simulink model "FullFMS_2026_02_18_V0_3_9"  (R2025b)
settings: Solver=ode23tb  StartTime=0.0  StopTime=inf  MaxStep=0.1  RelTol=1e-2
PreLoadFcn:
  | load("BUS_CONFIG.mat")
libraries: opcualib x8
(part 1 of 4)
settings Model: SimulationMode=accelerator  PacingRate=0.100000  Creator=guilh  LastModifiedBy=guilh
settings SolverCC: ZeroCrossControl=DisableAll

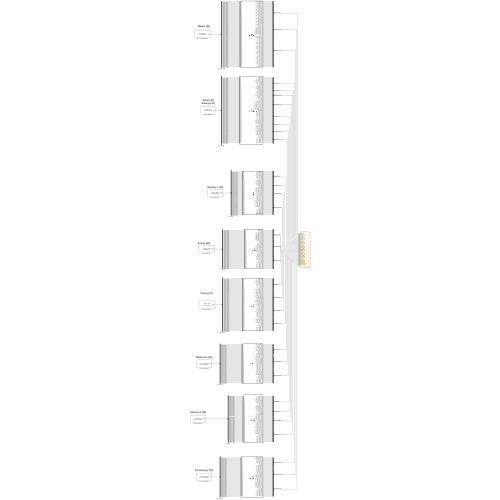
[thumbnail: Simulink's stored preview of the top-level diagram]
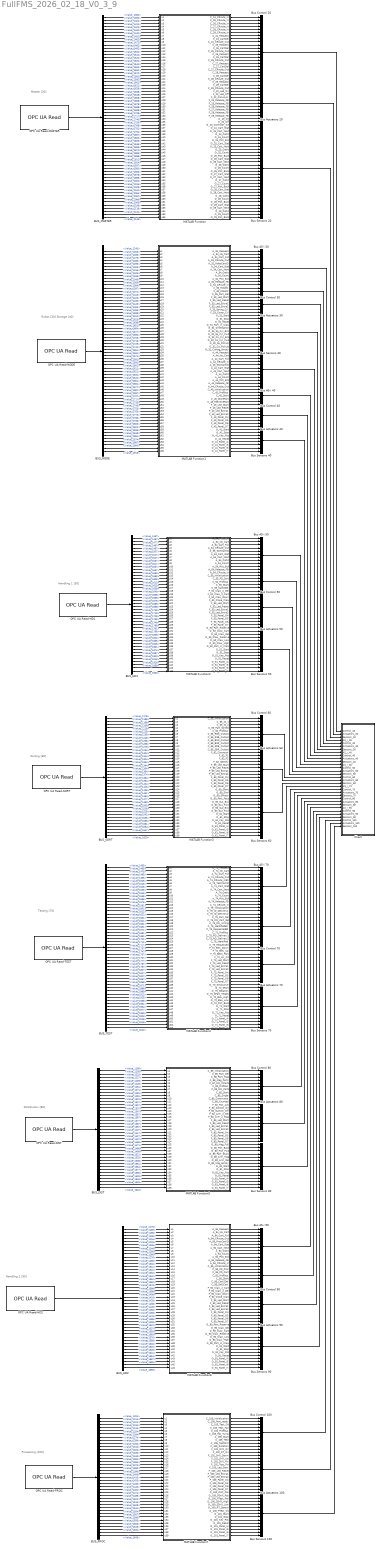
== system FullFMS_2026_02_18_V0_3_9 ==
  note: Master [20]
  note: Robot [30]
      | Storage [40]
  note: Handling 1 [50]
  note: Sorting [60]
  note: Testing [70]
  note: Distribution [80]
  note: Handling 2 [90]
  note: Processing [100]
  BUS_DIST : BusSelector  OutputSignals=Value_1195,Value_1205,Value_1215,Value_1227,Value_1239,Value_1249,Value_1261,Value_1271,Value_1281,Value_1291,Value_1301,Value_1317,Value_1327,Value_1337,Value_1347,Value_1357,Value_1367,Value_1377,Value_1387,Value_1397,Value_1407,Value_1417,Value_1427,Value_1437,Value_1458,Value_1471,Value_1486,Value_1499,Value_1512,Value_1525,Value_1538,Value_1551,Value_1564,Value_1577,Value_1590,Value_1603,Value_1616,Value_1629,Value_1642
  BUS_HD1 : BusSelector  OutputSignals=Value_1457,Value_1467,Value_1477,Value_1487,Value_1497,Value_1507,Value_1517,Value_1527,Value_1537,Value_1547,Value_1557,Value_1567,Value_1583,Value_1593,Value_1603,Value_1613,Value_1623,Value_1639,Value_1649,Value_1659,Value_1669,Value_1679,Value_1689,Value_1699,Value_1709,Value_1719,Value_1729,Value_1739,Value_1749,Value_1768,Value_1781,Value_1796,Value_1809,Value_1822,Value_1835,Value_1848,Value_1861,Value_1874,Value_1887,Value_1900,Value_1913,Value_1926,Value_1939,Value_1952
  BUS_HD2 : BusSelector  OutputSignals=Value_1176,Value_1186,Value_1196,Value_1206,Value_1216,Value_1226,Value_1236,Value_1246,Value_1256,Value_1266,Value_1276,Value_1286,Value_1302,Value_1312,Value_1322,Value_1332,Value_1342,Value_1352,Value_1362,Value_1378,Value_1388,Value_1398,Value_1408,Value_1418,Value_1428,Value_1438,Value_1448,Value_1458,Value_1468,Value_1478,Value_1488,Value_1509,Value_1522,Value_1537,Value_1550,Value_1563,Value_1576,Value_1589,Value_1602,Value_1615,Value_1628,Value_1641,Value_1654,Value_1667,Value_1680,Value_1693
  BUS_MASTER : BusSelector  OutputSignals=Value_1382,Value_1392,Value_1402,Value_1412,Value_1422,Value_1432,Value_1442,Value_1452,Value_1462,Value_1472,Value_1482,Value_1492,Value_1502,Value_1512,Value_1522,Value_1532,Value_1542,Value_1552,Value_1562,Value_1572,Value_1582,Value_1592,Value_1602,Value_1612,Value_1628,Value_1638,Value_1648,Value_1658,Value_1668,Value_1678,Value_1688,Value_1698,Value_1708,Value_1727,Value_1740,Value_1755,Value_1768,Value_1781,Value_1794,Value_1807,Value_1820,Value_1833,Value_1846,Value_1859,Value_1872,Value_1885,Value_1898,Value_1911,Value_1924,Value_1937,Value_1950,Value_1963,Value_1976,Value_1989,Value_2002,Value_2015,Value_2028,Value_2041,Value_2054,Value_2067,Value_2080,Value_2093,Value_2106,Value_2119,Value_2132,Value_2145
  BUS_NODE : BusSelector  OutputSignals=Value_1245,Value_1255,Value_1265,Value_1275,Value_1285,Value_1295,Value_1305,Value_1315,Value_1325,Value_1335,Value_1345,Value_1355,Value_1384,Value_1397,Value_1371,Value_1413,Value_1423,Value_1433,Value_1443,Value_1453,Value_1463,Value_1599,Value_1612,Value_1625,Value_1638,Value_1651,Value_1664,Value_1677,Value_1690,Value_1703,Value_1716,Value_1729,Value_1742,Value_2551,Value_2561,Value_2571,Value_2581,Value_2591,Value_2601,Value_2611,Value_2621,Value_2631,Value_2641,Value_2651,Value_2661,Value_2677,Value_2687,Value_2697,Value_2707,Value_2717,Value_2733,Value_2743,Value_2753,Value_2763,Value_2773,Value_2783,Value_2793,Value_2803,Value_2822,Value_2835,Value_2848,Value_2861,Value_2874,Value_2887,Value_2900,Value_2913
  BUS_PROC : BusSelector  OutputSignals=Value_1204,Value_1214,Value_1224,Value_1234,Value_1244,Value_1254,Value_1264,Value_1274,Value_1284,Value_1294,Value_1310,Value_1320,Value_1330,Value_1340,Value_1350,Value_1360,Value_1370,Value_1380,Value_1390,Value_1400,Value_1410,Value_1420,Value_1430,Value_1440,Value_1461,Value_1474,Value_1489,Value_1502,Value_1515,Value_1528,Value_1541,Value_1554,Value_1567,Value_1580,Value_1593,Value_1606,Value_1619,Value_1632,Value_1645
  BUS_SORT : BusSelector  OutputSignals=Value_1178,Value_1188,Value_1198,Value_1208,Value_1218,Value_1228,Value_1238,Value_1248,Value_1258,Value_1268,Value_1278,Value_1294,Value_1304,Value_1314,Value_1324,Value_1334,Value_1344,Value_1354,Value_1364,Value_1374,Value_1384,Value_1394,Value_1404,Value_1423,Value_1436,Value_1451,Value_1464,Value_1477,Value_1490,Value_1503,Value_1516,Value_1529,Value_1542,Value_1555,Value_1568,Value_1581,Value_1594,Value_1607,Value_1620
  BUS_TEST : BusSelector  OutputSignals=Value_1455,Value_1465,Value_1475,Value_1485,Value_1495,Value_1505,Value_1515,Value_1525,Value_1535,Value_1545,Value_1555,Value_1565,Value_1575,Value_1591,Value_1601,Value_1611,Value_1621,Value_1631,Value_1641,Value_1651,Value_1661,Value_1671,Value_1681,Value_1691,Value_1701,Value_1711,Value_1727,Value_1737,Value_1747,Value_1757,Value_1767,Value_1777,Value_1787,Value_1797,Value_1807,Value_1817,Value_1827,Value_1837,Value_1858,Value_1871,Value_1886,Value_1899,Value_1912,Value_1925,Value_1938,Value_1951,Value_1964,Value_1977,Value_1990,Value_2003,Value_2016,Value_2029,Value_2042
  Bus AS-i 30 : BusCreator  Inputs=12  OutDataTypeStr=Bus: B_ASI_ROBOT  NonVirtualBus=on
  Bus AS-i 40 : BusCreator  Inputs=12  OutDataTypeStr=Bus: B_ASI_STORAGE  NonVirtualBus=on
  Bus AS-i 50 : BusCreator  Inputs=12  OutDataTypeStr=Bus: B_ASI_HD1  NonVirtualBus=on
  Bus AS-i 70 : BusCreator  Inputs=13  OutDataTypeStr=Bus: B_ASI_TEST  NonVirtualBus=on
  Bus AS-i 90 : BusCreator  Inputs=12  OutDataTypeStr=Bus: B_ASI_HD2  NonVirtualBus=on
  Bus Actuators 100 : BusCreator  Inputs=14  OutDataTypeStr=Bus: B_F_PROC  NonVirtualBus=on
  Bus Actuators 20 : BusCreator  Inputs=9  OutDataTypeStr=Bus: B_F_MASTER  NonVirtualBus=on
  Bus Actuators 30 : BusCreator  Inputs=6  OutDataTypeStr=Bus: B_F_ROBOT  NonVirtualBus=on
  Bus Actuators 40 : BusCreator  Inputs=8  OutDataTypeStr=Bus: B_F_STORAGE  NonVirtualBus=on
  Bus Actuators 50 : BusCreator  Inputs=12  OutDataTypeStr=Bus: B_F_HD1  NonVirtualBus=on
  Bus Actuators 60 : BusCreator  Inputs=12  OutDataTypeStr=Bus: B_F_SORT  NonVirtualBus=on
  Bus Actuators 70 : BusCreator  Inputs=12  OutDataTypeStr=Bus: B_F_TEST  NonVirtualBus=on
  Bus Actuators 80 : BusCreator  Inputs=13  OutDataTypeStr=Bus: B_F_DIST  NonVirtualBus=on
  Bus Actuators 90 : BusCreator  Inputs=12  OutDataTypeStr=Bus: B_F_HD2  NonVirtualBus=on
  Bus Control 100 : BusCreator  Inputs=10  OutDataTypeStr=Bus: B_C_PROC  NonVirtualBus=on
  Bus Control 20 : BusCreator  Inputs=24  OutDataTypeStr=Bus: B_C_MASTER  NonVirtualBus=on
  Bus Control 30 : BusCreator  Inputs=3  OutDataTypeStr=Bus: B_C_ROBOT  NonVirtualBus=on
  Bus Control 40 : BusCreator  Inputs=5  OutDataTypeStr=Bus: B_C_STORAGE  NonVirtualBus=on
  Bus Control 50 : BusCreator  Inputs=5  OutDataTypeStr=Bus: B_C_HD1  NonVirtualBus=on
  Bus Control 60 : BusCreator  Inputs=11  OutDataTypeStr=Bus: B_C_SORT  NonVirtualBus=on
  Bus Control 70 : BusCreator  Inputs=13  OutDataTypeStr=Bus: B_C_TEST  NonVirtualBus=on
  Bus Control 80 : BusCreator  Inputs=11  OutDataTypeStr=Bus: B_C_DIST  NonVirtualBus=on
  Bus Control 90 : BusCreator  Inputs=7  OutDataTypeStr=Bus: B_C_HD2  NonVirtualBus=on
  Bus Sensors 100 : BusCreator  Inputs=15  OutDataTypeStr=Bus: B_S_PROC  NonVirtualBus=on
  Bus Sensors 20 : BusCreator  Inputs=33  OutDataTypeStr=Bus: B_S_MASTER  NonVirtualBus=on
  Bus Sensors 30 : BusCreator  Inputs=12  OutDataTypeStr=Bus: B_S_ROBOT  NonVirtualBus=on
  Bus Sensors 40 : BusCreator  Inputs=8  OutDataTypeStr=Bus: B_S_STORAGE  NonVirtualBus=on
  Bus Sensors 50 : BusCreator  Inputs=15  OutDataTypeStr=Bus: B_S_HD1  NonVirtualBus=on
  Bus Sensors 60 : BusCreator  Inputs=16  OutDataTypeStr=Bus: B_S_SORT  NonVirtualBus=on
  Bus Sensors 70 : BusCreator  Inputs=15  OutDataTypeStr=Bus: B_S_TEST  NonVirtualBus=on
  Bus Sensors 80 : BusCreator  Inputs=15  OutDataTypeStr=Bus: B_S_DIST  NonVirtualBus=on
  Bus Sensors 90 : BusCreator  Inputs=15  OutDataTypeStr=Bus: B_S_HD2  NonVirtualBus=on
  Chart : Stateflow chart  TreatAsAtomicUnit=on
      settings: PortSchema="{\"entries\":[{\"content\":{\"sides\":[{\"content\":{\"connectorIds\":[\"In18\",\"In12\",\"In24\",\"In8\",\"In19\",\"In13\",\"In25\",\"In30\",\"In29\",\"In31\",\"In32\",\"In9\",\"In20\",\"In14\",\"In26\",\"In21\",\"In15\",\"In27\",\"In4\",\"In5\",\"In6\",\"In7\",\"In1\",\"In2\",\"In3\",\"In10\",\"In22\",\"In16\",\"In28\",\"In17\",\"In11\",\"In23\"]},\"type\":\"ConnectorPlacement.EquallySpacedRectSide\",\"uuid\":\"e54bf7d4-7c7d-41d9-a8b8-f479ac319a99\"},{\"content\":{\"side\":\"RIGHT\"},\"type\":\"ConnectorPlacement.EquallySpacedRectSide\",\"uuid\":\"d3c20706-71bd-4e26-b40f-0ee7e71b06ee\"},{\"content\":{\"side\":\"TOP\"},\"type\":\"ConnectorPlacement.EquallySpacedRectSide\",\"uuid\":\"ecfb6920-e95b-4ed8-99f9-df5ce878328e\"}]},\"type\":\"ConnectorPlacement.EquallySpacedConnector\",\"uuid\":\"2e714192-4eea-4e1a-8945-7c827feed48f\"}],\"packageUris\":[\"http://schema.mathworks.com/mf0/Connector/R2020b\"],\"version\":\"1.0\"}"
  MATLAB Function : MATLAB Function  TreatAsAtomicUnit=on
  MATLAB Function1 : MATLAB Function  TreatAsAtomicUnit=on
  MATLAB Function2 : MATLAB Function  TreatAsAtomicUnit=on
  MATLAB Function3 : MATLAB Function  TreatAsAtomicUnit=on
  MATLAB Function4 : MATLAB Function  TreatAsAtomicUnit=on
  MATLAB Function5 : MATLAB Function  TreatAsAtomicUnit=on
  MATLAB Function6 : MATLAB Function  TreatAsAtomicUnit=on
  MATLAB Function7 : MATLAB Function  TreatAsAtomicUnit=on
  OPC UA Read-DIST : opcualib/OPC UA Read  SelectedServer=AAS OPC Distribution  ServerList=AAS OPC Distribution  NodeList={ '1','Value','6','1195','1'; '2','Value','6','1205','1'; '3','Value','6','1215','1'; '4','Value','6','1227','1'; '5','Value','6','1239','1'; '6','Value','6','1249','1'; '7','Value','6','1261','1'; '8','Value','6','1271','1'; '9','Value','6','1281','1'; '10','Value','6','1291','1'; '11','Value','6','1301','1'; '12','Value','6','1317','1'; '13','Value','6','1327','1'; '14','Value','6','1337','1'; '15','Value','6','1347','1'; '16','Value','6','1357','1'; '17','Value','6','1367','1'; '18','Value','6','1377','1'; '19','Value','6','1387','1'; '20','Value','6','1397','1'; '21','Value','6','1407','1'; '22','Value','6','1417','1'; '23','Value','6','1427','1'; '24','Value','6','1437','1'; '25','Value','6','1458','1'; '26','Value','6','1471','1'; '27','Value','6','1486','1'; '28','Value','6','1499','1'; '29','Value','6','1512','1'; '30','Value','6','1525','1'; '31','Value','6','1538','1'; '32','Value','6','1551','1'; '33','Value','6','1564','1'; '34','Value','6','1577','1'; '35','Value','6','1590','1'; '36','Value','6','1603','1'; '37','Value','6','1616','1'; '38','Value','6','1629','1'; '39','Value','6','1642','1' }  ShowQualityPort=off  ShowTimestampPort=off  ShowTimestampPortAs=Seconds since start  SampleTime=-1
  OPC UA Read-HD1 : opcualib/OPC UA Read  SelectedServer=AAS OPC Handling1  ServerList=AAS OPC Handling1  NodeList={ '1','Value','6','1457','1'; '2','Value','6','1467','1'; '3','Value','6','1477','1'; '4','Value','6','1487','1'; '5','Value','6','1497','1'; '6','Value','6','1507','1'; '7','Value','6','1517','1'; '8','Value','6','1527','1'; '9','Value','6','1537','1'; '10','Value','6','1547','1'; '11','Value','6','1557','1'; '12','Value','6','1567','1'; '13','Value','6','1583','1'; '14','Value','6','1593','1'; '15','Value','6','1603','1'; '16','Value','6','1613','1'; '17','Value','6','1623','1'; '18','Value','6','1639','1'; '19','Value','6','1649','1'; '20','Value','6','1659','1'; '21','Value','6','1669','1'; '22','Value','6','1679','1'; '23','Value','6','1689','1'; '24','Value','6','1699','1'; '25','Value','6','1709','1'; '26','Value','6','1719','1'; '27','Value','6','1729','1'; '28','Value','6','1739','1'; '29','Value','6','1749','1'; '30','Value','6','1768','1'; '31','Value','6','1781','1'; '32','Value','6','1796','1'; '33','Value','6','1809','1'; '34','Value','6','1822','1'; '35','Value','6','1835','1'; '36','Value','6','1848','1'; '37','Value','6','1861','1'; '38','Value','6','1874','1'; '39','Value','6','1887','1'; '40','Value','6','1900','1'; '41','Value','6','1913','1'; '42','Value','6','1926','1'; '43','Value','6','1939','1'; '44','Value','6','1952','1' }  ShowQualityPort=off  ShowTimestampPort=off  ShowTimestampPortAs=Seconds since start  SampleTime=-1
  OPC UA Read-HD2 : opcualib/OPC UA Read  SelectedServer=AAS OPC Handling2  ServerList=AAS OPC Handling2  NodeList={ '1','Value','6','1176','1'; '2','Value','6','1186','1'; '3','Value','6','1196','1'; '4','Value','6','1206','1'; '5','Value','6','1216','1'; '6','Value','6','1226','1'; '7','Value','6','1236','1'; '8','Value','6','1246','1'; '9','Value','6','1256','1'; '10','Value','6','1266','1'; '11','Value','6','1276','1'; '12','Value','6','1286','1'; '13','Value','6','1302','1'; '14','Value','6','1312','1'; '15','Value','6','1322','1'; '16','Value','6','1332','1'; '17','Value','6','1342','1'; '18','Value','6','1352','1'; '19','Value','6','1362','1'; '20','Value','6','1378','1'; '21','Value','6','1388','1'; '22','Value','6','1398','1'; '23','Value','6','1408','1'; '24','Value','6','1418','1'; '25','Value','6','1428','1'; '26','Value','6','1438','1'; '27','Value','6','1448','1'; '28','Value','6','1458','1'; '29','Value','6','1468','1'; '30','Value','6','1478','1'; '31','Value','6','1488','1'; '32','Value','6','1509','1'; '33','Value','6','1522','1'; '34','Value','6','1537','1'; '35','Value','6','1550','1'; '36','Value','6','1563','1'; '37','Value','6','1576','1'; '38','Value','6','1589','1'; '39','Value','6','1602','1'; '40','Value','6','1615','1'; '41','Value','6','1628','1'; '42','Value','6','1641','1'; '43','Value','6','1654','1'; '44','Value','6','1667','1'; '45','Value','6','1680','1'; '46','Value','6','1693','1' }  ShowQualityPort=off  ShowTimestampPort=off  ShowTimestampPortAs=Seconds since start  SampleTime=-1
  OPC UA Read-MASTER : opcualib/OPC UA Read  SelectedServer=AAS OPC Master  ServerList=AAS OPC Master  NodeList={ '1','Value','6','1382','1'; '2','Value','6','1392','1'; '3','Value','6','1402','1'; '4','Value','6','1412','1'; '5','Value','6','1422','1'; '6','Value','6','1432','1'; '7','Value','6','1442','1'; '8','Value','6','1452','1'; '9','Value','6','1462','1'; '10','Value','6','1472','1'; '11','Value','6','1482','1'; '12','Value','6','1492','1'; '13','Value','6','1502','1'; '14','Value','6','1512','1'; '15','Value','6','1522','1'; '16','Value','6','1532','1'; '17','Value','6','1542','1'; '18','Value','6','1552','1'; '19','Value','6','1562','1'; '20','Value','6','1572','1'; '21','Value','6','1582','1'; '22','Value','6','1592','1'; '23','Value','6','1602','1'; '24','Value','6','1612','1'; '25','Value','6','1628','1'; '26','Value','6','1638','1'; '27','Value','6','1648','1'; '28','Value','6','1658','1'; '29','Value','6','1668','1'; '30','Value','6','1678','1'; '31','Value','6','1688','1'; '32','Value','6','1698','1'; '33','Value','6','1708','1'; '34','Value','6','1727','1'; '35','Value','6','1740','1'; '36','Value','6','1755','1'; '37','Value','6','1768','1'; '38','Value','6','1781','1'; '39','Value','6','1794','1'; '40','Value','6','1807','1'; '41','Value','6','1820','1'; '42','Value','6','1833','1'; '43','Value','6','1846','1'; '44','Value','6','1859','1'; '45','Value','6','1872','1'; '46','Value','6','1885','1'; '47','Value','6','1898','1'; '48','Value','6','1911','1'; '49','Value','6','1924','1'; '50','Value','6','1937','1'; '51','Value','6','1950','1'; '52','Value','6','1963','1'; '53','Value','6','1976','1'; '54','Value','6','1989','1'; '55','Value','6','2002','1'; '56','Value','6','2015','1'; '57','Value','6','2028','1'; '58','Value','6','2041','1'; '59','Value','6','2054','1'; '60','Value','6','2067','1'; '61','Value','6','2080','1'; '62','Value','6','2093','1'; '63','Value','6','2106','1'; '64','Value','6','2119','1'; '65','Value','6','2132','1'; '66','Value','6','2145','1' }  ShowQualityPort=off  ShowTimestampPort=off  ShowTimestampPortAs=Seconds since start  SampleTime=-1
  OPC UA Read-NODE : opcualib/OPC UA Read  SelectedServer=Node-RED OPCUA  ServerList=Node-RED OPCUA  NodeList={ '1','Value','6','1245','1'; '2','Value','6','1255','1'; '3','Value','6','1265','1'; '4','Value','6','1275','1'; '5','Value','6','1285','1'; '6','Value','6','1295','1'; '7','Value','6','1305','1'; '8','Value','6','1315','1'; '9','Value','6','1325','1'; '10','Value','6','1335','1'; '11','Value','6','1345','1'; '12','Value','6','1355','1'; '13','Value','6','1384','1'; '14','Value','6','1397','1'; '15','Value','6','1371','1'; '16','Value','6','1413','1'; '17','Value','6','1423','1'; '18','Value','6','1433','1'; '19','Value','6','1443','1'; '20','Value','6','1453','1'; '21','Value','6','1463','1'; '22','Value','6','1599','1'; '23','Value','6','1612','1'; '24','Value','6','1625','1'; '25','Value','6','1638','1'; '26','Value','6','1651','1'; '27','Value','6','1664','1'; '28','Value','6','1677','1'; '29','Value','6','1690','1'; '30','Value','6','1703','1'; '31','Value','6','1716','1'; '32','Value','6','1729','1'; '33','Value','6','1742','1'; '34','Value','6','2551','1'; '35','Value','6','2561','1'; '36','Value','6','2571','1'; '37','Value','6','2581','1'; '38','Value','6','2591','1'; '39','Value','6','2601','1'; '40','Value','6','2611','1'; '41','Value','6','2621','1'; '42','Value','6','2631','1'; '43','Value','6','2641','1'; '44','Value','6','2651','1'; '45','Value','6','2661','1'; '46','Value','6','2677','1'; '47','Value','6','2687','1'; '48','Value','6','2697','1'; '49','Value','6','2707','1'; '50','Value','6','2717','1'; '51','Value','6','2733','1'; '52','Value','6','2743','1'; '53','Value','6','2753','1'; '54','Value','6','2763','1'; '55','Value','6','2773','1'; '56','Value','6','2783','1'; '57','Value','6','2793','1'; '58','Value','6','2803','1'; '59','Value','6','2822','1'; '60','Value','6','2835','1'; '61','Value','6','2848','1'; '62','Value','6','2861','1'; '63','Value','6','2874','1'; '64','Value','6','2887','1'; '65','Value','6','2900','1'; '66','Value','6','2913','1' }  ShowQualityPort=off  ShowTimestampPort=off  ShowTimestampPortAs=Seconds since start  SampleTime=-1
  OPC UA Read-PROC : opcualib/OPC UA Read  SelectedServer=AAS OPC Processing  ServerList=AAS OPC Processing  NodeList={ '1','Value','6','1204','1'; '2','Value','6','1214','1'; '3','Value','6','1224','1'; '4','Value','6','1234','1'; '5','Value','6','1244','1'; '6','Value','6','1254','1'; '7','Value','6','1264','1'; '8','Value','6','1274','1'; '9','Value','6','1284','1'; '10','Value','6','1294','1'; '11','Value','6','1310','1'; '12','Value','6','1320','1'; '13','Value','6','1330','1'; '14','Value','6','1340','1'; '15','Value','6','1350','1'; '16','Value','6','1360','1'; '17','Value','6','1370','1'; '18','Value','6','1380','1'; '19','Value','6','1390','1'; '20','Value','6','1400','1'; '21','Value','6','1410','1'; '22','Value','6','1420','1'; '23','Value','6','1430','1'; '24','Value','6','1440','1'; '25','Value','6','1461','1'; '26','Value','6','1474','1'; '27','Value','6','1489','1'; '28','Value','6','1502','1'; '29','Value','6','1515','1'; '30','Value','6','1528','1'; '31','Value','6','1541','1'; '32','Value','6','1554','1'; '33','Value','6','1567','1'; '34','Value','6','1580','1'; '35','Value','6','1593','1'; '36','Value','6','1606','1'; '37','Value','6','1619','1'; '38','Value','6','1632','1'; '39','Value','6','1645','1' }  ShowQualityPort=off  ShowTimestampPort=off  ShowTimestampPortAs=Seconds since start  SampleTime=-1
  OPC UA Read-SORT : opcualib/OPC UA Read  SelectedServer=AAS OPC Sorting  ServerList=AAS OPC Sorting  NodeList={ '1','Value','6','1178','1'; '2','Value','6','1188','1'; '3','Value','6','1198','1'; '4','Value','6','1208','1'; '5','Value','6','1218','1'; '6','Value','6','1228','1'; '7','Value','6','1238','1'; '8','Value','6','1248','1'; '9','Value','6','1258','1'; '10','Value','6','1268','1'; '11','Value','6','1278','1'; '12','Value','6','1294','1'; '13','Value','6','1304','1'; '14','Value','6','1314','1'; '15','Value','6','1324','1'; '16','Value','6','1334','1'; '17','Value','6','1344','1'; '18','Value','6','1354','1'; '19','Value','6','1364','1'; '20','Value','6','1374','1'; '21','Value','6','1384','1'; '22','Value','6','1394','1'; '23','Value','6','1404','1'; '24','Value','6','1423','1'; '25','Value','6','1436','1'; '26','Value','6','1451','1'; '27','Value','6','1464','1'; '28','Value','6','1477','1'; '29','Value','6','1490','1'; '30','Value','6','1503','1'; '31','Value','6','1516','1'; '32','Value','6','1529','1'; '33','Value','6','1542','1'; '34','Value','6','1555','1'; '35','Value','6','1568','1'; '36','Value','6','1581','1'; '37','Value','6','1594','1'; '38','Value','6','1607','1'; '39','Value','6','1620','1' }  ShowQualityPort=off  ShowTimestampPort=off  ShowTimestampPortAs=Seconds since start  SampleTime=-1
  OPC UA Read-TEST : opcualib/OPC UA Read  SelectedServer=AAS OPC Testing  ServerList=AAS OPC Testing  NodeList={ '1','Value','6','1455','1'; '2','Value','6','1465','1'; '3','Value','6','1475','1'; '4','Value','6','1485','1'; '5','Value','6','1495','1'; '6','Value','6','1505','1'; '7','Value','6','1515','1'; '8','Value','6','1525','1'; '9','Value','6','1535','1'; '10','Value','6','1545','1'; '11','Value','6','1555','1'; '12','Value','6','1565','1'; '13','Value','6','1575','1'; '14','Value','6','1591','1'; '15','Value','6','1601','1'; '16','Value','6','1611','1'; '17','Value','6','1621','1'; '18','Value','6','1631','1'; '19','Value','6','1641','1'; '20','Value','6','1651','1'; '21','Value','6','1661','1'; '22','Value','6','1671','1'; '23','Value','6','1681','1'; '24','Value','6','1691','1'; '25','Value','6','1701','1'; '26','Value','6','1711','1'; '27','Value','6','1727','1'; '28','Value','6','1737','1'; '29','Value','6','1747','1'; '30','Value','6','1757','1'; '31','Value','6','1767','1'; '32','Value','6','1777','1'; '33','Value','6','1787','1'; '34','Value','6','1797','1'; '35','Value','6','1807','1'; '36','Value','6','1817','1'; '37','Value','6','1827','1'; '38','Value','6','1837','1'; '39','Value','6','1858','1'; '40','Value','6','1871','1'; '41','Value','6','1886','1'; '42','Value','6','1899','1'; '43','Value','6','1912','1'; '44','Value','6','1925','1'; '45','Value','6','1938','1'; '46','Value','6','1951','1'; '47','Value','6','1964','1'; '48','Value','6','1977','1'; '49','Value','6','1990','1'; '50','Value','6','2003','1'; '51','Value','6','2016','1'; '52','Value','6','2029','1'; '53','Value','6','2042','1' }  ShowQualityPort=off  ShowTimestampPort=off  ShowTimestampPortAs=Seconds since start  SampleTime=-1
  wires:
  MATLAB Function5/12(F_82_Pist_Adv) -> Bus Actuators 80/1
  MATLAB Function5/13(F_82_Suction_On) -> Bus Actuators 80/2
  MATLAB Function5/14(F_82_Suction_Off) -> Bus Actuators 80/3
  MATLAB Function5/15(F_82_Arm_2_Del) -> Bus Actuators 80/4
  MATLAB Function5/16(F_82_Arm_2_Mag) -> Bus Actuators 80/5
  MATLAB Function5/17(F_83_Led_Start) -> Bus Actuators 80/6
  MATLAB Function5/18(F_83_Led_Reset) -> Bus Actuators 80/7
  MATLAB Function5/19(F_83_Led_Extra1) -> Bus Actuators 80/8
  MATLAB Function5/20(F_83_Led_Extra2) -> Bus Actuators 80/9
  MATLAB Function5/21(F_83_Panel_O4) -> Bus Actuators 80/10
  MATLAB Function5/22(F_83_Panel_O5) -> Bus Actuators 80/11
  MATLAB Function5/23(F_83_Panel_O6) -> Bus Actuators 80/12
  MATLAB Function5/24(F_83_Panel_O7) -> Bus Actuators 80/13
  MATLAB Function5/25(O_80_Mag_Full) -> Bus Sensors 80/1
  MATLAB Function5/26(O_80_Pist_Back) -> Bus Sensors 80/2
  MATLAB Function5/27(O_80_Pist_Fwd) -> Bus Sensors 80/3
  MATLAB Function5/28(O_80_Part_Stuck) -> Bus Sensors 80/4
  MATLAB Function5/29(O_80_Arm_Mag) -> Bus Sensors 80/5
  MATLAB Function5/30(O_80_Arm_Del) -> Bus Sensors 80/6
  MATLAB Function5/31(O_80_Mag_Empty) -> Bus Sensors 80/7
  MATLAB Function5/32(O_81_Start) -> Bus Sensors 80/8
  MATLAB Function5/33(O_81_Stop) -> Bus Sensors 80/9
  MATLAB Function5/34(O_81_Key_Pos) -> Bus Sensors 80/10
  MATLAB Function5/35(O_81_Reset) -> Bus Sensors 80/11
  MATLAB Function5/36(O_81_Panel_I4) -> Bus Sensors 80/12
  MATLAB Function5/37(O_81_Panel_I5) -> Bus Sensors 80/13
  MATLAB Function5/38(O_81_Panel_I6) -> Bus Sensors 80/14
  MATLAB Function5/39(O_81_Panel_I7) -> Bus Sensors 80/15
  MATLAB Function4/1(A_74_Request) -> Bus AS-i 70/1
  MATLAB Function4/2(A_74_No_Cart) -> Bus AS-i 70/2
  MATLAB Function4/3(A_74_Cart_Full) -> Bus AS-i 70/3
  MATLAB Function4/4(A_74_CRoute_Out) -> Bus AS-i 70/4
  MATLAB Function4/5(A_74_CRoute_In80) -> Bus AS-i 70/5
  MATLAB Function4/6(A_73_TestCartID) -> Bus AS-i 70/6
  MATLAB Function4/7(A_74_Cart_Stat) -> Bus AS-i 70/7
  MATLAB Function4/8(A_74_Cart_Next) -> Bus AS-i 70/8
  MATLAB Function4/9(A_74_Optic) -> Bus AS-i 70/9
  MATLAB Function4/10(A_74_Count) -> Bus AS-i 70/10
  MATLAB Function4/11(A_74_Pist_Bck) -> Bus AS-i 70/11
  MATLAB Function4/12(A_74_Release_FB) -> Bus AS-i 70/12
  MATLAB Function4/13(A_74_CRoute_In) -> Bus AS-i 70/13
  MATLAB Function4/14(C_75_Initialization) -> Bus Control 70/1
  MATLAB Function4/15(C_75_ID_Delivery1) -> Bus Control 70/2
  MATLAB Function4/16(C_75_ID_Delivery2) -> Bus Control 70/3
  MATLAB Function4/17(C_75_Part_Del) -> Bus Control 70/4
  MATLAB Function4/18(C_75_RQ_Part_Del) -> Bus Control 70/5
  MATLAB Function4/19(C_75_RQ_Wrong) -> Bus Control 70/6
  MATLAB Function4/20(C_75_Identified80) -> Bus Control 70/7
  MATLAB Function4/21(C_75_Requested80) -> Bus Control 70/8
  MATLAB Function4/22(C_72_Profibus) -> Bus Control 70/9
  MATLAB Function4/23(C_75_RQ_Delivery1) -> Bus Control 70/10
  MATLAB Function4/24(C_75_RQ_Delivery2) -> Bus Control 70/11
  MATLAB Function4/25(C_75_Identified) -> Bus Control 70/12
  MATLAB Function4/26(C_75_Requested) -> Bus Control 70/13
  MATLAB Function4/27(F_72_Elev_Down) -> Bus Actuators 70/1
  MATLAB Function4/28(F_72_Elev_Up) -> Bus Actuators 70/2
  MATLAB Function4/29(F_72_Eject_Part) -> Bus Actuators 70/3
  MATLAB Function4/30(F_72_Air_On) -> Bus Actuators 70/4
  MATLAB Function4/31(F_73_Led_Start) -> Bus Actuators 70/5
  MATLAB Function4/32(F_73_Led_Reset) -> Bus Actuators 70/6
  MATLAB Function4/33(F_73_Led_Extra1) -> Bus Actuators 70/7
  MATLAB Function4/34(F_73_Led_Extra2) -> Bus Actuators 70/8
  MATLAB Function4/35(F_73_Panel_O4) -> Bus Actuators 70/9
  MATLAB Function4/36(F_73_Panel_O5) -> Bus Actuators 70/10
  MATLAB Function4/37(F_73_Panel_O6) -> Bus Actuators 70/11
  MATLAB Function4/38(F_73_Panel_O7) -> Bus Actuators 70/12
  MATLAB Function4/39(O_70_SInductive) -> Bus Sensors 70/1
  MATLAB Function4/40(O_70_SPart) -> Bus Sensors 70/2
  MATLAB Function4/41(O_70_SStation) -> Bus Sensors 70/3
  MATLAB Function4/42(O_70_SPart_Height) -> Bus Sensors 70/4
  MATLAB Function4/43(O_70_Elev_High) -> Bus Sensors 70/5
  MATLAB Function4/44(O_70_Elev_Low) -> Bus Sensors 70/6
  MATLAB Function4/45(O_70_Pist_Back) -> Bus Sensors 70/7
  MATLAB Function4/46(O_71_Start) -> Bus Sensors 70/8
  MATLAB Function4/47(O_71_Stop) -> Bus Sensors 70/9
  MATLAB Function4/48(O_71_Key_Pos) -> Bus Sensors 70/10
  MATLAB Function4/49(O_71_Reset) -> Bus Sensors 70/11
  MATLAB Function4/50(O_71_Panel_I4) -> Bus Sensors 70/12
  MATLAB Function4/51(O_71_Panel_I5) -> Bus Sensors 70/13
  MATLAB Function4/52(O_71_Panel_I6) -> Bus Sensors 70/14
  MATLAB Function4/53(O_71_Panel_I7) -> Bus Sensors 70/15
  Bus Control 80/1 -> Chart/1(Control_80)
  Bus Actuators 80/1 -> Chart/2(Actuators_80)
  Bus Sensors 80/1 -> Chart/3(Sensors_80)
  Bus Sensors 70/1 -> Chart/7(Sensors_70)
  Bus Actuators 70/1 -> Chart/6(Actuators_70)
  Bus Control 70/1 -> Chart/5(Control_70)
  Bus AS-i 70/1 -> Chart/4(AS_i_70)
  MATLAB Function/1(C_24_CRoute_In) -> Bus Control 20/1
  MATLAB Function/2(C_25_CRoute_In) -> Bus Control 20/2
  MATLAB Function/3(C_26_CRoute_In) -> Bus Control 20/3
  MATLAB Function/4(C_27_CRoute_In) -> Bus Control 20/4
  MATLAB Function/5(C_28_CRoute_In) -> Bus Control 20/5
  MATLAB Function/6(C_29_CRoute_In) -> Bus Control 20/6
  MATLAB Function/7(C_24_Request) -> Bus Control 20/7
  MATLAB Function/8(C_24_CartDel) -> Bus Control 20/8
  MATLAB Function/9(C_24_CRoute_Out) -> Bus Control 20/9
  MATLAB Function/10(C_25_Request) -> Bus Control 20/10
  MATLAB Function/11(C_25_CartDel) -> Bus Control 20/11
  MATLAB Function/12(C_25_CRoute_Out) -> Bus Control 20/12
  MATLAB Function/13(C_26_Request) -> Bus Control 20/13
  MATLAB Function/14(C_26_CartDel) -> Bus Control 20/14
  MATLAB Function/15(C_26_CRoute_Out) -> Bus Control 20/15
  MATLAB Function/16(C_27_Request) -> Bus Control 20/16
  MATLAB Function/17(C_27_CartDel) -> Bus Control 20/17
  MATLAB Function/18(C_27_CRoute_Out) -> Bus Control 20/18
  MATLAB Function/19(C_28_Request) -> Bus Control 20/19
  MATLAB Function/20(C_28_CartDel) -> Bus Control 20/20
  MATLAB Function/21(C_28_CRoute_Out) -> Bus Control 20/21
  MATLAB Function/22(C_29_Request) -> Bus Control 20/22
  MATLAB Function/23(C_29_CartDel) -> Bus Control 20/23
  MATLAB Function/24(C_29_CRoute_Out) -> Bus Control 20/24
  MATLAB Function/25(F_22_Led_On) -> Bus Actuators 20/1
  MATLAB Function/26(F_22_Led_Off) -> Bus Actuators 20/2
  MATLAB Function/27(F_22_Conveyor) -> Bus Actuators 20/3
  MATLAB Function/28(F_24_Release_FB) -> Bus Actuators 20/4
  MATLAB Function/29(F_25_Release_FB) -> Bus Actuators 20/5
  MATLAB Function/30(F_26_Release_FB) -> Bus Actuators 20/6
  MATLAB Function/31(F_27_Release_FB) -> Bus Actuators 20/7
  MATLAB Function/32(F_28_Release_FB) -> Bus Actuators 20/8
  MATLAB Function/33(F_29_Release_FB) -> Bus Actuators 20/9
  MATLAB Function/34(O_20_On) -> Bus Sensors 20/1
  MATLAB Function/35(O_20_Off) -> Bus Sensors 20/2
  MATLAB Function/36(O_20_Controler_On) -> Bus Sensors 20/3
  MATLAB Function/37(O_24_Cart_Stat) -> Bus Sensors 20/4
  MATLAB Function/38(O_24_Cart_Next) -> Bus Sensors 20/5
  MATLAB Function/39(O_24_Optic) -> Bus Sensors 20/6
  MATLAB Function/40(O_24_Count) -> Bus Sensors 20/7
  MATLAB Function/41(O_24_Pist_Bck) -> Bus Sensors 20/8
  MATLAB Function/42(O_25_Cart_Stat) -> Bus Sensors 20/9
  MATLAB Function/43(O_25_Cart_Next) -> Bus Sensors 20/10
  MATLAB Function/44(O_25_Optic) -> Bus Sensors 20/11
  MATLAB Function/45(O_25_Count) -> Bus Sensors 20/12
  MATLAB Function/46(O_25_Pist_Back) -> Bus Sensors 20/13
  MATLAB Function/47(O_26_Cart_Stat) -> Bus Sensors 20/14
  MATLAB Function/48(O_26_Cart_Next) -> Bus Sensors 20/15
  MATLAB Function/49(O_26_Optic) -> Bus Sensors 20/16
  MATLAB Function/50(O_26_Count) -> Bus Sensors 20/17
  MATLAB Function/51(O_26_Pist_Back) -> Bus Sensors 20/18
  MATLAB Function/52(O_27_Cart_Stat) -> Bus Sensors 20/19
  MATLAB Function/53(O_27_Cart_Next) -> Bus Sensors 20/20
  MATLAB Function/54(O_27_Optic) -> Bus Sensors 20/21
  MATLAB Function/55(O_27_Count) -> Bus Sensors 20/22
  MATLAB Function/56(O_27_Pist_Back) -> Bus Sensors 20/23
  MATLAB Function/57(O_28_Cart_Stat) -> Bus Sensors 20/24
  MATLAB Function/58(O_28_Cart_Next) -> Bus Sensors 20/25
  MATLAB Function/59(O_28_Optic) -> Bus Sensors 20/26
  MATLAB Function/60(O_28_Count) -> Bus Sensors 20/27
  MATLAB Function/61(O_28_Pist_Back) -> Bus Sensors 20/28
  MATLAB Function/62(O_29_Cart_Stat) -> Bus Sensors 20/29
  MATLAB Function/63(O_29_Cart_Next) -> Bus Sensors 20/30
  MATLAB Function/64(O_29_Optic) -> Bus Sensors 20/31
  MATLAB Function/65(O_29_Count) -> Bus Sensors 20/32
  MATLAB Function/66(O_29_Pist_Back) -> Bus Sensors 20/33
  Bus Control 20/1 -> Chart/18(Control_20)
  Bus Actuators 20/1 -> Chart/12(Actuators_20)
  Bus Sensors 20/1 -> Chart/24(Sensors_20)
  MATLAB Function2/30(O_50_Part_Reserve) -> Bus Sensors 50/1
  MATLAB Function2/31(O_50_Claw_Cart) -> Bus Sensors 50/2
  MATLAB Function2/32(O_50_Claw_Del) -> Bus Sensors 50/3
  MATLAB Function2/33(O_50_Claw_Reserve) -> Bus Sensors 50/4
  MATLAB Function2/34(O_50_Claw_Low) -> Bus Sensors 50/5
  MATLAB Function2/35(O_50_Claw_High) -> Bus Sensors 50/6
  MATLAB Function2/36(O_50_Part_in_Claw) -> Bus Sensors 50/7
  MATLAB Function2/37(O_51_Start) -> Bus Sensors 50/8
  MATLAB Function2/38(O_51_Stop) -> Bus Sensors 50/9
  MATLAB Function2/39(O_51_Key_Pos) -> Bus Sensors 50/10
  MATLAB Function2/40(O_51_Reset) -> Bus Sensors 50/11
  MATLAB Function2/41(O_51_Panel_I4) -> Bus Sensors 50/12
  MATLAB Function2/42(O_51_Panel_I5) -> Bus Sensors 50/13
  MATLAB Function2/43(O_51_Panel_I6) -> Bus Sensors 50/14
  MATLAB Function2/44(O_51_Panel_I7) -> Bus Sensors 50/15
  MATLAB Function2/18(F_52_Claw_2_Del) -> Bus Actuators 50/1
  MATLAB Function2/19(F_52_Claw_2_Cart) -> Bus Actuators 50/2
  MATLAB Function2/20(F_52_Claw_Down) -> Bus Actuators 50/3
  MATLAB Function2/21(F_52_Close_Claw) -> Bus Actuators 50/4
  MATLAB Function2/22(F_53_Led_Start) -> Bus Actuators 50/5
  MATLAB Function2/23(F_53_Led_Reset) -> Bus Actuators 50/6
  MATLAB Function2/24(F_53_Led_Extra1) -> Bus Actuators 50/7
  MATLAB Function2/25(F_53_Led_Extra2) -> Bus Actuators 50/8
  MATLAB Function2/26(F_53_Panel_O4) -> Bus Actuators 50/9
  MATLAB Function2/27(F_53_Panel_O5) -> Bus Actuators 50/10
  MATLAB Function2/28(F_53_Panel_O6) -> Bus Actuators 50/11
  MATLAB Function2/29(F_53_Panel_O7) -> Bus Actuators 50/12
  MATLAB Function2/13(C_55_Initialization) -> Bus Control 50/1
  MATLAB Function2/14(C_55_PD_Sort) -> Bus Control 50/2
  MATLAB Function2/15(C_52_Profibus) -> Bus Control 50/3
  MATLAB Function2/16(C_55_Start) -> Bus Control 50/4
  MATLAB Function2/17(C_55_Cart2Del) -> Bus Control 50/5
  Bus AS-i 50/1 -> Chart/9(AS_i_50)
  Bus Control 50/1 -> Chart/20(Control_50)
  Bus Actuators 50/1 -> Chart/14(Actuators_50)
  Bus Sensors 50/1 -> Chart/26(Sensors_50)
  MATLAB Function6/1(A_94_Request) -> Bus AS-i 90/1
  MATLAB Function6/2(A_94_No_Cart) -> Bus AS-i 90/2
  MATLAB Function6/3(A_94_Cart_Full) -> Bus AS-i 90/3
  MATLAB Function6/4(A_94_CRoute_Out) -> Bus AS-i 90/4
  MATLAB Function6/5(A_93_ProcCartID) -> Bus AS-i 90/5
  MATLAB Function6/6(A_94_Cart_Stat) -> Bus AS-i 90/6
  MATLAB Function6/7(A_94_Cart_Next) -> Bus AS-i 90/7
  MATLAB Function6/8(A_94_Optic) -> Bus AS-i 90/8
  MATLAB Function6/9(A_94_Count) -> Bus AS-i 90/9
  MATLAB Function6/10(A_94_Pist_Bck) -> Bus AS-i 90/10
  MATLAB Function6/11(A_94_Release_FB) -> Bus AS-i 90/11
  MATLAB Function6/12(A_94_CRoute_In) -> Bus AS-i 90/12
  MATLAB Function6/13(C_95_Initialization) -> Bus Control 90/1
  MATLAB Function6/14(C_95_PD_Proc) -> Bus Control 90/2
  MATLAB Function6/15(C_95_PD_Cart) -> Bus Control 90/3
  MATLAB Function6/16(C_92_Profibus) -> Bus Control 90/4
  MATLAB Function6/17(C_95_Start) -> Bus Control 90/5
  MATLAB Function6/18(C_95_Cart2Del) -> Bus Control 90/6
  MATLAB Function6/19(C_95_Del2Cart) -> Bus Control 90/7
  MATLAB Function6/20(F_92_Claw_2_Cart) -> Bus Actuators 90/1
  MATLAB Function6/21(F_92_Claw_2_Del) -> Bus Actuators 90/2
  MATLAB Function6/22(F_92_Claw_Down) -> Bus Actuators 90/3
  MATLAB Function6/23(F_92_Close_Claw) -> Bus Actuators 90/4
  MATLAB Function6/24(F_93_Led_Start) -> Bus Actuators 90/5
  MATLAB Function6/25(F_93_Led_Reset) -> Bus Actuators 90/6
  MATLAB Function6/26(F_93_Led_Extra1) -> Bus Actuators 90/7
  MATLAB Function6/27(F_93_Led_Extra2) -> Bus Actuators 90/8
  MATLAB Function6/28(F_93_Panel_O4) -> Bus Actuators 90/9
  MATLAB Function6/29(F_93_Panel_O5) -> Bus Actuators 90/10
  MATLAB Function6/30(F_93_Panel_O6) -> Bus Actuators 90/11
  MATLAB Function6/31(F_93_Panel_O7) -> Bus Actuators 90/12
  MATLAB Function6/32(O_90_Part_Reserve) -> Bus Sensors 90/1
  MATLAB Function6/33(O_90_Claw_Del) -> Bus Sensors 90/2
  MATLAB Function6/34(O_90_Claw_Cart) -> Bus Sensors 90/3
  MATLAB Function6/35(O_90_Claw_Reserve) -> Bus Sensors 90/4
  MATLAB Function6/36(O_90_Claw_Low) -> Bus Sensors 90/5
  MATLAB Function6/37(O_90_Claw_High) -> Bus Sensors 90/6
  MATLAB Function6/38(O_90_Part_in_Claw) -> Bus Sensors 90/7
  MATLAB Function6/39(O_91_Start) -> Bus Sensors 90/8
  MATLAB Function6/40(O_91_Stop) -> Bus Sensors 90/9
  MATLAB Function6/41(O_91_Key_Pos) -> Bus Sensors 90/10
  MATLAB Function6/42(O_91_Reset) -> Bus Sensors 90/11
  MATLAB Function6/43(O_91_Panel_I4) -> Bus Sensors 90/12
  MATLAB Function6/44(O_91_Panel_I5) -> Bus Sensors 90/13
  MATLAB Function6/45(O_91_Panel_I6) -> Bus Sensors 90/14
  MATLAB Function6/46(O_91_Panel_I7) -> Bus Sensors 90/15
  Bus AS-i 90/1 -> Chart/10(AS_i_90)
  Bus Control 90/1 -> Chart/22(Control_90)
  Bus Actuators 90/1 -> Chart/16(Actuators_90)
  Bus Sensors 90/1 -> Chart/28(Sensors_90)
  MATLAB Function7/25(O_100_PInit_Pos) -> Bus Sensors 100/1
  MATLAB Function7/26(O_100_PDrill_Pos) -> Bus Sensors 100/2
  MATLAB Function7/27(O_100_PTest_Pos) -> Bus Sensors 100/3
  MATLAB Function7/28(O_100_SDrill_High) -> Bus Sensors 100/4
  MATLAB Function7/29(O_100_SDrill_Low) -> Bus Sensors 100/5
  MATLAB Function7/30(O_100_RT_Sensor) -> Bus Sensors 100/6
  MATLAB Function7/31(O_100_PTest_Ok) -> Bus Sensors 100/7
  MATLAB Function7/32(O_101_Start) -> Bus Sensors 100/8
  MATLAB Function7/33(O_101_Stop) -> Bus Sensors 100/9
  MATLAB Function7/34(O_101_Key_Pos) -> Bus Sensors 100/10
  MATLAB Function7/35(O_101_Reset) -> Bus Sensors 100/11
  MATLAB Function7/36(O_101_Panel_I4) -> Bus Sensors 100/12
  MATLAB Function7/37(O_101_Panel_I5) -> Bus Sensors 100/13
  MATLAB Function7/38(O_101_Panel_I6) -> Bus Sensors 100/14
  MATLAB Function7/39(O_101_Panel_I7) -> Bus Sensors 100/15
  MATLAB Function7/1(C_105_Initialization) -> Bus Control 100/1
  MATLAB Function7/2(C_105_Part_ready) -> Bus Control 100/2
  MATLAB Function7/3(C_105_Test_Ok) -> Bus Control 100/3
  MATLAB Function7/4(C_105_Test_Fail) -> Bus Control 100/4
  MATLAB Function7/5(C_102_Profibus) -> Bus Control 100/5
  MATLAB Function7/6(C_103_RQ_Turns) -> Bus Control 100/6
  MATLAB Function7/7(C_105_Start) -> Bus Control 100/7
  MATLAB Function7/8(C_105_Test) -> Bus Control 100/8
  MATLAB Function7/9(C_105_TestDrill) -> Bus Control 100/9
  MATLAB Function7/10(C_105_Rotation) -> Bus Control 100/10
  MATLAB Function7/11(F_102_Drill_On) -> Bus Actuators 100/1
  MATLAB Function7/12(F_102_RT_On) -> Bus Actuators 100/2
  MATLAB Function7/13(F_102_Drill_Down) -> Bus Actuators 100/3
  MATLAB Function7/14(F_102_Drill_Up) -> Bus Actuators 100/4
  MATLAB Function7/15(F_102_Drill_Pin) -> Bus Actuators 100/5
  MATLAB Function7/16(F_102_Test_Pin) -> Bus Actuators 100/6
  MATLAB Function7/17(F_103_Led_Start) -> Bus Actuators 100/7
  MATLAB Function7/18(F_103_Led_Reset) -> Bus Actuators 100/8
  MATLAB Function7/19(F_103_Led_Extra1) -> Bus Actuators 100/9
  MATLAB Function7/20(F_103_Led_Extra2) -> Bus Actuators 100/10
  MATLAB Function7/21(F_103_Panel_O4) -> Bus Actuators 100/11
  MATLAB Function7/22(F_103_Panel_O5) -> Bus Actuators 100/12
  MATLAB Function7/23(F_103_Panel_O6) -> Bus Actuators 100/13
  MATLAB Function7/24(F_103_Panel_O7) -> Bus Actuators 100/14
  Bus Control 100/1 -> Chart/17(Control_100)
  Bus Actuators 100/1 -> Chart/11(Actuators_100)
  Bus Sensors 100/1 -> Chart/23(Sensors_100)
  MATLAB Function1/1(A_34_Request) -> Bus AS-i 30/1
  MATLAB Function1/2(A_34_No_Cart) -> Bus AS-i 30/2
  MATLAB Function1/3(A_34_Cart_Full) -> Bus AS-i 30/3
  MATLAB Function1/4(A_34_CRoute_Out) -> Bus AS-i 30/4
  MATLAB Function1/5(A_32_RoboCartID) -> Bus AS-i 30/5
  MATLAB Function1/6(A_34_Cart_Stat) -> Bus AS-i 30/6
  MATLAB Function1/7(A_34_Cart_Next) -> Bus AS-i 30/7
  MATLAB Function1/8(A_34_Optic) -> Bus AS-i 30/8
  MATLAB Function1/9(A_34_Count) -> Bus AS-i 30/9
  MATLAB Function1/10(A_34_Pist_Bck) -> Bus AS-i 30/10
  MATLAB Function1/11(A_34_Release_FB) -> Bus AS-i 30/11
  MATLAB Function1/12(A_34_CRoute_In) -> Bus AS-i 30/12
  MATLAB Function1/16(F_33_Led_Start) -> Bus Actuators 30/1
  MATLAB Function1/17(F_33_Led_Reset) -> Bus Actuators 30/2
  MATLAB Function1/18(F_33_Led_Extra1) -> Bus Actuators 30/3
  MATLAB Function1/19(F_33_Led_Extra2) -> Bus Actuators 30/4
  MATLAB Function1/20(F_33_Spring_Cyl) -> Bus Actuators 30/5
  MATLAB Function1/21(F_33_Cover_Cyl) -> Bus Actuators 30/6
  MATLAB Function1/22(O_31_Start) -> Bus Sensors 30/1
  MATLAB Function1/23(O_31_Stop) -> Bus Sensors 30/2
  MATLAB Function1/24(O_31_Reset) -> Bus Sensors 30/3
  MATLAB Function1/25(O_31_Part_in_Claw) -> Bus Sensors 30/4
  MATLAB Function1/26(O_31_Orientation) -> Bus Sensors 30/5
  MATLAB Function1/27(O_32_Sp_Cyl_Bck) -> Bus Sensors 30/6
  MATLAB Function1/28(O_32_Sp_Cyl_Fwd) -> Bus Sensors 30/7
  MATLAB Function1/29(O_32_Co_Cyl_Bck) -> Bus Sensors 30/8
  MATLAB Function1/30(O_32_Co_Cyl_Fwd) -> Bus Sensors 30/9
  MATLAB Function1/31(O_32_Sp_PickUp) -> Bus Sensors 30/10
  MATLAB Function1/32(O_32_Co_PickUp) -> Bus Sensors 30/11
  MATLAB Function1/33(O_32_CoMag_Empty) -> Bus Sensors 30/12
  Bus AS-i 30/1 -> Chart/8(AS_i_30)
  Bus Control 30/1 -> Chart/19(Control_30)
  Bus Actuators 30/1 -> Chart/13(Actuators_30)
  Bus Sensors 30/1 -> Chart/25(Sensors_30)
  MATLAB Function3/1(C_65_Initialization) -> Bus Control 60/1
  MATLAB Function3/2(C_65_ID_1) -> Bus Control 60/2
  MATLAB Function3/3(C_65_ID_2) -> Bus Control 60/3
  MATLAB Function3/4(C_65_Part_Sorted) -> Bus Control 60/4
  MATLAB Function3/5(C_62_Profibus) -> Bus Control 60/5
  MATLAB Function3/6(C_65_RBS_Output) -> Bus Control 60/6
  MATLAB Function3/7(C_65_RSB_Output) -> Bus Control 60/7
  MATLAB Function3/8(C_65_BRS_Output) -> Bus Control 60/8
  MATLAB Function3/9(C_65_BSR_Output) -> Bus Control 60/9
  MATLAB Function3/10(C_65_SRB_Output) -> Bus Control 60/10
  MATLAB Function3/11(C_65_SBR_Output) -> Bus Control 60/11
  MATLAB Function3/12(F_62_Conveyor) -> Bus Actuators 60/1
  MATLAB Function3/13(F_62_P1) -> Bus Actuators 60/2
  MATLAB Function3/14(F_62_P2) -> Bus Actuators 60/3
  MATLAB Function3/15(F_62_Identify) -> Bus Actuators 60/4
  MATLAB Function3/16(F_63_Led_Start) -> Bus Actuators 60/5
  MATLAB Function3/17(F_63_Led_Reset) -> Bus Actuators 60/6
  MATLAB Function3/18(F_63_Led_Extra1) -> Bus Actuators 60/7
  MATLAB Function3/19(F_63_Led_Extra2) -> Bus Actuators 60/8
  MATLAB Function3/20(F_63_Panel_O4) -> Bus Actuators 60/9
  MATLAB Function3/21(F_63_Panel_O5) -> Bus Actuators 60/10
  MATLAB Function3/22(F_63_Panel_O6) -> Bus Actuators 60/11
  MATLAB Function3/23(F_63_Panel_O7) -> Bus Actuators 60/12
  MATLAB Function3/24(O_60_SPart) -> Bus Sensors 60/1
  MATLAB Function3/25(O_60_Slnd) -> Bus Sensors 60/2
  MATLAB Function3/26(O_60_SPhoto) -> Bus Sensors 60/3
  MATLAB Function3/27(O_60_Part_Pass) -> Bus Sensors 60/4
  MATLAB Function3/28(O_60_SL1_Bck) -> Bus Sensors 60/5
  MATLAB Function3/29(O_60_SL1_Fwd) -> Bus Sensors 60/6
  MATLAB Function3/30(O_60_SL2_Bck) -> Bus Sensors 60/7
  MATLAB Function3/31(O_60_SL2_Fwd) -> Bus Sensors 60/8
  MATLAB Function3/32(O_61_Start) -> Bus Sensors 60/9
  MATLAB Function3/33(O_61_Stop) -> Bus Sensors 60/10
  MATLAB Function3/34(O_61_Key_Pos) -> Bus Sensors 60/11
  MATLAB Function3/35(O_61_Reset) -> Bus Sensors 60/12
  MATLAB Function3/36(O_61_Panel_I4) -> Bus Sensors 60/13
  MATLAB Function3/37(O_61_Panel_I5) -> Bus Sensors 60/14
  MATLAB Function3/38(O_61_Panel_I6) -> Bus Sensors 60/15
  MATLAB Function3/39(O_61_Panel_I7) -> Bus Sensors 60/16
  Bus Control 60/1 -> Chart/21(Control_60)
  Bus Actuators 60/1 -> Chart/15(Actuators_60)
  Bus Sensors 60/1 -> Chart/27(Sensors_60)
  MATLAB Function1/46(C_45_Initialization) -> Bus Control 40/1
  MATLAB Function1/47(C_42_Profibus) -> Bus Control 40/2
  MATLAB Function1/48(C_45_Start) -> Bus Control 40/3
  MATLAB Function1/49(C_45_StorePart) -> Bus Control 40/4
  MATLAB Function1/50(C_45_RetrievePart) -> Bus Control 40/5
  MATLAB Function1/51(F_43_Led_Start) -> Bus Actuators 40/1
  MATLAB Function1/52(F_43_Led_Reset) -> Bus Actuators 40/2
  MATLAB Function1/53(F_43_Led_Extra1) -> Bus Actuators 40/3
  MATLAB Function1/54(F_43_Led_Extra2) -> Bus Actuators 40/4
  MATLAB Function1/55(F_43_Panel_O4) -> Bus Actuators 40/5
  MATLAB Function1/56(F_43_Panel_O5) -> Bus Actuators 40/6
  MATLAB Function1/57(F_43_Panel_O6) -> Bus Actuators 40/7
  MATLAB Function1/58(F_43_Panel_O7) -> Bus Actuators 40/8
  MATLAB Function1/59(O_41_Start) -> Bus Sensors 40/1
  MATLAB Function1/60(O_41_Stop) -> Bus Sensors 40/2
  MATLAB Function1/61(O_41_Key_Pos) -> Bus Sensors 40/3
  MATLAB Function1/62(O_41_Reset) -> Bus Sensors 40/4
  MATLAB Function1/63(O_41_Panel_I4) -> Bus Sensors 40/5
  MATLAB Function1/64(O_41_Panel_I5) -> Bus Sensors 40/6
  MATLAB Function1/65(O_41_Panel_I6) -> Bus Sensors 40/7
  MATLAB Function1/66(O_41_Panel_I7) -> Bus Sensors 40/8
  Bus AS-i 40/1 -> Chart/30(AS_i_40)
  Bus Control 40/1 -> Chart/29(Control_40)
  Bus Actuators 40/1 -> Chart/31(Actuators_40)
  Bus Sensors 40/1 -> Chart/32(Sensors_40)
  MATLAB Function5/1(C_85_Initialization) -> Bus Control 80/1
  MATLAB Function5/2(C_85_Part_Del) -> Bus Control 80/2
  MATLAB Function5/3(C_85_Part_Mag) -> Bus Control 80/3
  MATLAB Function5/4(C_86_Mag_Parts) -> Bus Control 80/4
  MATLAB Function5/5(C_87_RQ_MParts) -> Bus Control 80/5
  MATLAB Function5/6(C_82_Profibus) -> Bus Control 80/6
  MATLAB Function5/7(C_83_RQ_Parts) -> Bus Control 80/7
  MATLAB Function5/8(C_85_Start) -> Bus Control 80/8
  MATLAB Function5/9(C_85_Single) -> Bus Control 80/9
  MATLAB Function5/10(C_85_Continuous) -> Bus Control 80/10
  MATLAB Function5/11(C_85_Counted) -> Bus Control 80/11
  MATLAB Function2/1(A_54_Request) -> Bus AS-i 50/1
  MATLAB Function2/2(A_54_No_Cart) -> Bus AS-i 50/2
  MATLAB Function2/3(A_54_Cart_Full) -> Bus AS-i 50/3
  MATLAB Function2/4(A_54_CRoute_Out) -> Bus AS-i 50/4
  MATLAB Function2/5(A_53_SortCartID) -> Bus AS-i 50/5
  MATLAB Function2/6(A_54_Cart_Stat) -> Bus AS-i 50/6
  MATLAB Function2/7(A_54_Cart_Next) -> Bus AS-i 50/7
  MATLAB Function2/8(A_54_Optic) -> Bus AS-i 50/8
  MATLAB Function2/9(A_54_Count) -> Bus AS-i 50/9
  MATLAB Function2/10(A_54_Pist_Bck) -> Bus AS-i 50/10
  MATLAB Function2/11(A_54_Release_FB) -> Bus AS-i 50/11
  MATLAB Function2/12(A_54_CRoute_In) -> Bus AS-i 50/12
  MATLAB Function1/34(A_44_Request) -> Bus AS-i 40/1
  MATLAB Function1/35(A_44_No_Cart) -> Bus AS-i 40/2
  MATLAB Function1/36(A_44_Cart_Full) -> Bus AS-i 40/3
  MATLAB Function1/37(A_44_CRoute_In) -> Bus AS-i 40/4
  MATLAB Function1/38(A_43_StorCartID) -> Bus AS-i 40/5
  MATLAB Function1/39(A_44_Cart_Stat) -> Bus AS-i 40/6
  MATLAB Function1/40(A_44_Cart_Next) -> Bus AS-i 40/7
  MATLAB Function1/41(A_44_Optic) -> Bus AS-i 40/8
  MATLAB Function1/42(A_44_Count) -> Bus AS-i 40/9
  MATLAB Function1/43(A_44_Pist_Bck) -> Bus AS-i 40/10
  MATLAB Function1/44(A_44_Release_FB) -> Bus AS-i 40/11
  MATLAB Function1/45(A_44_CRoute_Out) -> Bus AS-i 40/12
  OPC UA Read-DIST/1 -> BUS_DIST/1
  OPC UA Read-MASTER/1 -> BUS_MASTER/1
  OPC UA Read-HD2/1 -> BUS_HD2/1
  OPC UA Read-PROC/1 -> BUS_PROC/1
  OPC UA Read-TEST/1 -> BUS_TEST/1
  OPC UA Read-SORT/1 -> BUS_SORT/1
  OPC UA Read-HD1/1 -> BUS_HD1/1
  OPC UA Read-NODE/1 -> BUS_NODE/1
  BUS_MASTER/1 -> MATLAB Function/1(u1)  "<Value_1382>"
  BUS_MASTER/2 -> MATLAB Function/2(u2)  "<Value_1392>"
  BUS_MASTER/3 -> MATLAB Function/3(u3)  "<Value_1402>"
  BUS_MASTER/4 -> MATLAB Function/4(u4)  "<Value_1412>"
  BUS_MASTER/5 -> MATLAB Function/5(u5)  "<Value_1422>"
  BUS_MASTER/6 -> MATLAB Function/6(u6)  "<Value_1432>"
  BUS_MASTER/7 -> MATLAB Function/7(u7)  "<Value_1442>"
  BUS_MASTER/8 -> MATLAB Function/8(u8)  "<Value_1452>"
  BUS_MASTER/9 -> MATLAB Function/9(u9)  "<Value_1462>"
  BUS_MASTER/10 -> MATLAB Function/10(u10)  "<Value_1472>"
  BUS_MASTER/11 -> MATLAB Function/11(u11)  "<Value_1482>"
  BUS_MASTER/12 -> MATLAB Function/12(u12)  "<Value_1492>"
  BUS_MASTER/13 -> MATLAB Function/13(u13)  "<Value_1502>"
  BUS_MASTER/14 -> MATLAB Function/14(u14)  "<Value_1512>"
  BUS_MASTER/15 -> MATLAB Function/15(u15)  "<Value_1522>"
  BUS_MASTER/16 -> MATLAB Function/16(u16)  "<Value_1532>"
  BUS_MASTER/17 -> MATLAB Function/17(u17)  "<Value_1542>"
  BUS_MASTER/18 -> MATLAB Function/18(u18)  "<Value_1552>"
  BUS_MASTER/19 -> MATLAB Function/19(u19)  "<Value_1562>"
  BUS_MASTER/20 -> MATLAB Function/20(u20)  "<Value_1572>"
  BUS_MASTER/21 -> MATLAB Function/21(u21)  "<Value_1582>"
  BUS_MASTER/22 -> MATLAB Function/22(u22)  "<Value_1592>"
  BUS_MASTER/23 -> MATLAB Function/23(u23)  "<Value_1602>"
  BUS_MASTER/24 -> MATLAB Function/24(u24)  "<Value_1612>"
  BUS_MASTER/25 -> MATLAB Function/25(u25)  "<Value_1628>"
  BUS_MASTER/26 -> MATLAB Function/26(u26)  "<Value_1638>"
  BUS_MASTER/27 -> MATLAB Function/27(u27)  "<Value_1648>"
  BUS_MASTER/28 -> MATLAB Function/28(u28)  "<Value_1658>"
  BUS_MASTER/29 -> MATLAB Function/29(u29)  "<Value_1668>"
  BUS_MASTER/30 -> MATLAB Function/30(u30)  "<Value_1678>"
  BUS_MASTER/31 -> MATLAB Function/31(u31)  "<Value_1688>"
  BUS_MASTER/32 -> MATLAB Function/32(u32)  "<Value_1698>"
  BUS_MASTER/33 -> MATLAB Function/33(u33)  "<Value_1708>"
  BUS_MASTER/34 -> MATLAB Function/34(u34)  "<Value_1727>"
  BUS_MASTER/35 -> MATLAB Function/35(u35)  "<Value_1740>"
  BUS_MASTER/36 -> MATLAB Function/36(u36)  "<Value_1755>"
  BUS_MASTER/37 -> MATLAB Function/37(u37)  "<Value_1768>"
  BUS_MASTER/38 -> MATLAB Function/38(u38)  "<Value_1781>"
  BUS_MASTER/39 -> MATLAB Function/39(u39)  "<Value_1794>"
  BUS_MASTER/40 -> MATLAB Function/40(u40)  "<Value_1807>"
  BUS_MASTER/41 -> MATLAB Function/41(u41)  "<Value_1820>"
  BUS_MASTER/42 -> MATLAB Function/42(u42)  "<Value_1833>"
  BUS_MASTER/43 -> MATLAB Function/43(u43)  "<Value_1846>"
  BUS_MASTER/44 -> MATLAB Function/44(u44)  "<Value_1859>"
  BUS_MASTER/45 -> MATLAB Function/45(u45)  "<Value_1872>"
  BUS_MASTER/46 -> MATLAB Function/46(u46)  "<Value_1885>"
  BUS_MASTER/47 -> MATLAB Function/47(u47)  "<Value_1898>"
  BUS_MASTER/48 -> MATLAB Function/48(u48)  "<Value_1911>"
  BUS_MASTER/49 -> MATLAB Function/49(u49)  "<Value_1924>"
  BUS_MASTER/50 -> MATLAB Function/50(u50)  "<Value_1937>"
  BUS_MASTER/51 -> MATLAB Function/51(u51)  "<Value_1950>"
  BUS_MASTER/52 -> MATLAB Function/52(u52)  "<Value_1963>"
  BUS_MASTER/53 -> MATLAB Function/53(u53)  "<Value_1976>"
  BUS_MASTER/54 -> MATLAB Function/54(u54)  "<Value_1989>"
  BUS_MASTER/55 -> MATLAB Function/55(u55)  "<Value_2002>"
  BUS_MASTER/56 -> MATLAB Function/56(u56)  "<Value_2015>"
  BUS_MASTER/57 -> MATLAB Function/57(u57)  "<Value_2028>"
  BUS_MASTER/58 -> MATLAB Function/58(u58)  "<Value_2041>"
  BUS_MASTER/59 -> MATLAB Function/59(u59)  "<Value_2054>"
  BUS_MASTER/60 -> MATLAB Function/60(u60)  "<Value_2067>"
  BUS_MASTER/61 -> MATLAB Function/61(u61)  "<Value_2080>"
  BUS_MASTER/62 -> MATLAB Function/62(u62)  "<Value_2093>"
  BUS_MASTER/63 -> MATLAB Function/63(u63)  "<Value_2106>"
  BUS_MASTER/64 -> MATLAB Function/64(u64)  "<Value_2119>"
  BUS_MASTER/65 -> MATLAB Function/65(u65)  "<Value_2132>"
  BUS_MASTER/66 -> MATLAB Function/66(u66)  "<Value_2145>"
  MATLAB Function1/13(C_30_Robot1) -> Bus Control 30/1
  MATLAB Function1/14(C_30_Robot2) -> Bus Control 30/2
  MATLAB Function1/15(C_35_Part_Del) -> Bus Control 30/3
  BUS_HD1/1 -> MATLAB Function2/1(u1)  "<Value_1457>"
  BUS_HD1/2 -> MATLAB Function2/2(u2)  "<Value_1467>"
  BUS_HD1/3 -> MATLAB Function2/3(u3)  "<Value_1477>"
  BUS_HD1/4 -> MATLAB Function2/4(u4)  "<Value_1487>"
  BUS_HD1/5 -> MATLAB Function2/5(u5)  "<Value_1497>"
  BUS_HD1/6 -> MATLAB Function2/6(u6)  "<Value_1507>"
  BUS_HD1/7 -> MATLAB Function2/7(u7)  "<Value_1517>"
  BUS_HD1/8 -> MATLAB Function2/8(u8)  "<Value_1527>"
  BUS_HD1/9 -> MATLAB Function2/9(u9)  "<Value_1537>"
  BUS_HD1/10 -> MATLAB Function2/10(u10)  "<Value_1547>"
  BUS_HD1/11 -> MATLAB Function2/11(u11)  "<Value_1557>"
  BUS_HD1/12 -> MATLAB Function2/12(u12)  "<Value_1567>"
  BUS_HD1/13 -> MATLAB Function2/13(u13)  "<Value_1583>"
  BUS_HD1/14 -> MATLAB Function2/14(u14)  "<Value_1593>"
  BUS_HD1/15 -> MATLAB Function2/15(u15)  "<Value_1603>"
  BUS_HD1/16 -> MATLAB Function2/16(u16)  "<Value_1613>"
  BUS_HD1/17 -> MATLAB Function2/17(u17)  "<Value_1623>"
  BUS_HD1/18 -> MATLAB Function2/18(u18)  "<Value_1639>"
  BUS_HD1/19 -> MATLAB Function2/19(u19)  "<Value_1649>"
  BUS_HD1/20 -> MATLAB Function2/20(u20)  "<Value_1659>"
  BUS_HD1/21 -> MATLAB Function2/21(u21)  "<Value_1669>"
  BUS_HD1/22 -> MATLAB Function2/22(u22)  "<Value_1679>"
  BUS_HD1/23 -> MATLAB Function2/23(u23)  "<Value_1689>"
  BUS_HD1/24 -> MATLAB Function2/24(u24)  "<Value_1699>"
  BUS_HD1/25 -> MATLAB Function2/25(u25)  "<Value_1709>"
  BUS_HD1/26 -> MATLAB Function2/26(u26)  "<Value_1719>"
  BUS_HD1/27 -> MATLAB Function2/27(u27)  "<Value_1729>"
  BUS_HD1/28 -> MATLAB Function2/28(u28)  "<Value_1739>"
  BUS_HD1/29 -> MATLAB Function2/29(u29)  "<Value_1749>"
  BUS_HD1/30 -> MATLAB Function2/30(u30)  "<Value_1768>"
  BUS_HD1/31 -> MATLAB Function2/31(u31)  "<Value_1781>"
  BUS_HD1/32 -> MATLAB Function2/32(u32)  "<Value_1796>"
  BUS_HD1/33 -> MATLAB Function2/33(u33)  "<Value_1809>"
  BUS_HD1/34 -> MATLAB Function2/34(u34)  "<Value_1822>"
  BUS_HD1/35 -> MATLAB Function2/35(u35)  "<Value_1835>"
  BUS_HD1/36 -> MATLAB Function2/36(u36)  "<Value_1848>"
  BUS_HD1/37 -> MATLAB Function2/37(u37)  "<Value_1861>"
  BUS_HD1/38 -> MATLAB Function2/38(u38)  "<Value_1874>"
  BUS_HD1/39 -> MATLAB Function2/39(u39)  "<Value_1887>"
  BUS_HD1/40 -> MATLAB Function2/40(u40)  "<Value_1900>"
  BUS_HD1/41 -> MATLAB Function2/41(u41)  "<Value_1913>"
  BUS_HD1/42 -> MATLAB Function2/42(u42)  "<Value_1926>"
  BUS_HD1/43 -> MATLAB Function2/43(u43)  "<Value_1939>"
  BUS_HD1/44 -> MATLAB Function2/44(u44)  "<Value_1952>"
  BUS_SORT/1 -> MATLAB Function3/1(u1)  "<Value_1178>"
  BUS_SORT/2 -> MATLAB Function3/2(u2)  "<Value_1188>"
  BUS_SORT/3 -> MATLAB Function3/3(u3)  "<Value_1198>"
  BUS_SORT/4 -> MATLAB Function3/4(u4)  "<Value_1208>"
  BUS_SORT/5 -> MATLAB Function3/5(u5)  "<Value_1218>"
  BUS_SORT/6 -> MATLAB Function3/6(u6)  "<Value_1228>"
  BUS_SORT/7 -> MATLAB Function3/7(u7)  "<Value_1238>"
  BUS_SORT/8 -> MATLAB Function3/8(u8)  "<Value_1248>"
  BUS_SORT/9 -> MATLAB Function3/9(u9)  "<Value_1258>"
  BUS_SORT/10 -> MATLAB Function3/10(u10)  "<Value_1268>"
  BUS_SORT/11 -> MATLAB Function3/11(u11)  "<Value_1278>"
  BUS_SORT/12 -> MATLAB Function3/12(u12)  "<Value_1294>"
  BUS_SORT/13 -> MATLAB Function3/13(u13)  "<Value_1304>"
  BUS_SORT/14 -> MATLAB Function3/14(u14)  "<Value_1314>"
  BUS_SORT/15 -> MATLAB Function3/15(u15)  "<Value_1324>"
  BUS_SORT/16 -> MATLAB Function3/16(u16)  "<Value_1334>"
  BUS_SORT/17 -> MATLAB Function3/17(u17)  "<Value_1344>"
  BUS_SORT/18 -> MATLAB Function3/18(u18)  "<Value_1354>"
  BUS_SORT/19 -> MATLAB Function3/19(u19)  "<Value_1364>"
  BUS_SORT/20 -> MATLAB Function3/20(u20)  "<Value_1374>"
  BUS_SORT/21 -> MATLAB Function3/21(u21)  "<Value_1384>"
  BUS_SORT/22 -> MATLAB Function3/22(u22)  "<Value_1394>"
  BUS_SORT/23 -> MATLAB Function3/23(u23)  "<Value_1404>"
  BUS_SORT/24 -> MATLAB Function3/24(u24)  "<Value_1423>"
  BUS_SORT/25 -> MATLAB Function3/25(u25)  "<Value_1436>"
  BUS_SORT/26 -> MATLAB Function3/26(u26)  "<Value_1451>"
  BUS_SORT/27 -> MATLAB Function3/27(u27)  "<Value_1464>"
  BUS_SORT/28 -> MATLAB Function3/28(u28)  "<Value_1477>"
  BUS_SORT/29 -> MATLAB Function3/29(u29)  "<Value_1490>"
  BUS_SORT/30 -> MATLAB Function3/30(u30)  "<Value_1503>"
  BUS_SORT/31 -> MATLAB Function3/31(u31)  "<Value_1516>"
  BUS_SORT/32 -> MATLAB Function3/32(u32)  "<Value_1529>"
  BUS_SORT/33 -> MATLAB Function3/33(u33)  "<Value_1542>"
  BUS_SORT/34 -> MATLAB Function3/34(u34)  "<Value_1555>"
  BUS_SORT/35 -> MATLAB Function3/35(u35)  "<Value_1568>"
  BUS_SORT/36 -> MATLAB Function3/36(u36)  "<Value_1581>"
  BUS_SORT/37 -> MATLAB Function3/37(u37)  "<Value_1594>"
  BUS_SORT/38 -> MATLAB Function3/38(u38)  "<Value_1607>"
  BUS_SORT/39 -> MATLAB Function3/39(u39)  "<Value_1620>"
  BUS_TEST/1 -> MATLAB Function4/1(u1)  "<Value_1455>"
  BUS_TEST/2 -> MATLAB Function4/2(u2)  "<Value_1465>"
  BUS_TEST/3 -> MATLAB Function4/3(u3)  "<Value_1475>"
  BUS_TEST/4 -> MATLAB Function4/4(u4)  "<Value_1485>"
  BUS_TEST/5 -> MATLAB Function4/5(u5)  "<Value_1495>"
  BUS_TEST/6 -> MATLAB Function4/6(u6)  "<Value_1505>"
  BUS_TEST/7 -> MATLAB Function4/7(u7)  "<Value_1515>"
  BUS_TEST/8 -> MATLAB Function4/8(u8)  "<Value_1525>"
  BUS_TEST/9 -> MATLAB Function4/9(u9)  "<Value_1535>"
  BUS_TEST/10 -> MATLAB Function4/10(u10)  "<Value_1545>"
  BUS_TEST/11 -> MATLAB Function4/11(u11)  "<Value_1555>"
  BUS_TEST/12 -> MATLAB Function4/12(u12)  "<Value_1565>"
  BUS_TEST/13 -> MATLAB Function4/13(u13)  "<Value_1575>"
  BUS_TEST/14 -> MATLAB Function4/14(u14)  "<Value_1591>"
  BUS_TEST/15 -> MATLAB Function4/15(u15)  "<Value_1601>"
  BUS_TEST/16 -> MATLAB Function4/16(u16)  "<Value_1611>"
  BUS_TEST/17 -> MATLAB Function4/17(u17)  "<Value_1621>"
  BUS_TEST/18 -> MATLAB Function4/18(u18)  "<Value_1631>"
  BUS_TEST/19 -> MATLAB Function4/19(u19)  "<Value_1641>"
  BUS_TEST/20 -> MATLAB Function4/20(u20)  "<Value_1651>"
  BUS_TEST/21 -> MATLAB Function4/21(u21)  "<Value_1661>"
  BUS_TEST/22 -> MATLAB Function4/22(u22)  "<Value_1671>"
  BUS_TEST/23 -> MATLAB Function4/23(u23)  "<Value_1681>"
  BUS_TEST/24 -> MATLAB Function4/24(u24)  "<Value_1691>"
  BUS_TEST/25 -> MATLAB Function4/25(u25)  "<Value_1701>"
  BUS_TEST/26 -> MATLAB Function4/26(u26)  "<Value_1711>"
  BUS_TEST/27 -> MATLAB Function4/27(u27)  "<Value_1727>"
  BUS_TEST/28 -> MATLAB Function4/28(u28)  "<Value_1737>"
  BUS_TEST/29 -> MATLAB Function4/29(u29)  "<Value_1747>"
  BUS_TEST/30 -> MATLAB Function4/30(u30)  "<Value_1757>"
  BUS_TEST/31 -> MATLAB Function4/31(u31)  "<Value_1767>"
  BUS_TEST/32 -> MATLAB Function4/32(u32)  "<Value_1777>"
  BUS_TEST/33 -> MATLAB Function4/33(u33)  "<Value_1787>"
  BUS_TEST/34 -> MATLAB Function4/34(u34)  "<Value_1797>"
  BUS_TEST/35 -> MATLAB Function4/35(u35)  "<Value_1807>"
  BUS_TEST/36 -> MATLAB Function4/36(u36)  "<Value_1817>"
  BUS_TEST/37 -> MATLAB Function4/37(u37)  "<Value_1827>"
  BUS_TEST/38 -> MATLAB Function4/38(u38)  "<Value_1837>"
  BUS_TEST/39 -> MATLAB Function4/39(u39)  "<Value_1858>"
  BUS_TEST/40 -> MATLAB Function4/40(u40)  "<Value_1871>"
  BUS_TEST/41 -> MATLAB Function4/41(u41)  "<Value_1886>"
  BUS_TEST/42 -> MATLAB Function4/42(u42)  "<Value_1899>"
  BUS_TEST/43 -> MATLAB Function4/43(u43)  "<Value_1912>"
  BUS_TEST/44 -> MATLAB Function4/44(u44)  "<Value_1925>"
  BUS_TEST/45 -> MATLAB Function4/45(u45)  "<Value_1938>"
  BUS_TEST/46 -> MATLAB Function4/46(u46)  "<Value_1951>"
  BUS_TEST/47 -> MATLAB Function4/47(u47)  "<Value_1964>"
  BUS_TEST/48 -> MATLAB Function4/48(u48)  "<Value_1977>"
  BUS_TEST/49 -> MATLAB Function4/49(u49)  "<Value_1990>"
  BUS_TEST/50 -> MATLAB Function4/50(u50)  "<Value_2003>"
  BUS_TEST/51 -> MATLAB Function4/51(u51)  "<Value_2016>"
  BUS_TEST/52 -> MATLAB Function4/52(u52)  "<Value_2029>"
  BUS_TEST/53 -> MATLAB Function4/53(u53)  "<Value_2042>"
  BUS_DIST/1 -> MATLAB Function5/1(u1)  "<Value_1195>"
  BUS_DIST/2 -> MATLAB Function5/2(u2)  "<Value_1205>"
  BUS_DIST/3 -> MATLAB Function5/3(u3)  "<Value_1215>"
  BUS_DIST/4 -> MATLAB Function5/4(u4)  "<Value_1227>"
  BUS_DIST/5 -> MATLAB Function5/5(u5)  "<Value_1239>"
  BUS_DIST/6 -> MATLAB Function5/6(u6)  "<Value_1249>"
  BUS_DIST/7 -> MATLAB Function5/7(u7)  "<Value_1261>"
  BUS_DIST/8 -> MATLAB Function5/8(u8)  "<Value_1271>"
  BUS_DIST/9 -> MATLAB Function5/9(u9)  "<Value_1281>"
  BUS_DIST/10 -> MATLAB Function5/10(u10)  "<Value_1291>"
  BUS_DIST/11 -> MATLAB Function5/11(u11)  "<Value_1301>"
  BUS_DIST/12 -> MATLAB Function5/12(u12)  "<Value_1317>"
  BUS_DIST/13 -> MATLAB Function5/13(u13)  "<Value_1327>"
  BUS_DIST/14 -> MATLAB Function5/14(u14)  "<Value_1337>"
  BUS_DIST/15 -> MATLAB Function5/15(u15)  "<Value_1347>"
  BUS_DIST/16 -> MATLAB Function5/16(u16)  "<Value_1357>"
  BUS_DIST/17 -> MATLAB Function5/17(u17)  "<Value_1367>"
  BUS_DIST/18 -> MATLAB Function5/18(u18)  "<Value_1377>"
  BUS_DIST/19 -> MATLAB Function5/19(u19)  "<Value_1387>"
  BUS_DIST/20 -> MATLAB Function5/20(u20)  "<Value_1397>"
  BUS_DIST/21 -> MATLAB Function5/21(u21)  "<Value_1407>"
  BUS_DIST/22 -> MATLAB Function5/22(u22)  "<Value_1417>"
  BUS_DIST/23 -> MATLAB Function5/23(u23)  "<Value_1427>"
  BUS_DIST/24 -> MATLAB Function5/24(u24)  "<Value_1437>"
  BUS_DIST/25 -> MATLAB Function5/25(u25)  "<Value_1458>"
  BUS_DIST/26 -> MATLAB Function5/26(u26)  "<Value_1471>"
  BUS_DIST/27 -> MATLAB Function5/27(u27)  "<Value_1486>"
  BUS_DIST/28 -> MATLAB Function5/28(u28)  "<Value_1499>"
  BUS_DIST/29 -> MATLAB Function5/29(u29)  "<Value_1512>"
  BUS_DIST/30 -> MATLAB Function5/30(u30)  "<Value_1525>"
  BUS_DIST/31 -> MATLAB Function5/31(u31)  "<Value_1538>"
  BUS_DIST/32 -> MATLAB Function5/32(u32)  "<Value_1551>"
  BUS_DIST/33 -> MATLAB Function5/33(u33)  "<Value_1564>"
  BUS_DIST/34 -> MATLAB Function5/34(u34)  "<Value_1577>"
  BUS_DIST/35 -> MATLAB Function5/35(u35)  "<Value_1590>"
  BUS_DIST/36 -> MATLAB Function5/36(u36)  "<Value_1603>"
  BUS_DIST/37 -> MATLAB Function5/37(u37)  "<Value_1616>"
  BUS_DIST/38 -> MATLAB Function5/38(u38)  "<Value_1629>"
  BUS_DIST/39 -> MATLAB Function5/39(u39)  "<Value_1642>"
  BUS_HD2/1 -> MATLAB Function6/1(u1)  "<Value_1176>"
  BUS_HD2/2 -> MATLAB Function6/2(u2)  "<Value_1186>"
  BUS_HD2/3 -> MATLAB Function6/3(u3)  "<Value_1196>"
  BUS_HD2/4 -> MATLAB Function6/4(u4)  "<Value_1206>"
  BUS_HD2/5 -> MATLAB Function6/5(u5)  "<Value_1216>"
  BUS_HD2/6 -> MATLAB Function6/6(u6)  "<Value_1226>"
  BUS_HD2/7 -> MATLAB Function6/7(u7)  "<Value_1236>"
  BUS_HD2/8 -> MATLAB Function6/8(u8)  "<Value_1246>"
  BUS_HD2/9 -> MATLAB Function6/9(u9)  "<Value_1256>"
  BUS_HD2/10 -> MATLAB Function6/10(u10)  "<Value_1266>"
  BUS_HD2/11 -> MATLAB Function6/11(u11)  "<Value_1276>"
  BUS_HD2/12 -> MATLAB Function6/12(u12)  "<Value_1286>"
  BUS_HD2/13 -> MATLAB Function6/13(u13)  "<Value_1302>"
  BUS_HD2/14 -> MATLAB Function6/14(u14)  "<Value_1312>"
  BUS_HD2/15 -> MATLAB Function6/15(u15)  "<Value_1322>"
  BUS_HD2/16 -> MATLAB Function6/16(u16)  "<Value_1332>"
  BUS_HD2/17 -> MATLAB Function6/17(u17)  "<Value_1342>"
  BUS_HD2/18 -> MATLAB Function6/18(u18)  "<Value_1352>"
  BUS_HD2/19 -> MATLAB Function6/19(u19)  "<Value_1362>"
  BUS_HD2/20 -> MATLAB Function6/20(u20)  "<Value_1378>"
  BUS_HD2/21 -> MATLAB Function6/21(u21)  "<Value_1388>"
  BUS_HD2/22 -> MATLAB Function6/22(u22)  "<Value_1398>"
  BUS_HD2/23 -> MATLAB Function6/23(u23)  "<Value_1408>"
  BUS_HD2/24 -> MATLAB Function6/24(u24)  "<Value_1418>"
  BUS_HD2/25 -> MATLAB Function6/25(u25)  "<Value_1428>"
  BUS_HD2/26 -> MATLAB Function6/26(u26)  "<Value_1438>"
  BUS_HD2/27 -> MATLAB Function6/27(u27)  "<Value_1448>"
  BUS_HD2/28 -> MATLAB Function6/28(u28)  "<Value_1458>"
  BUS_HD2/29 -> MATLAB Function6/29(u29)  "<Value_1468>"
  BUS_HD2/30 -> MATLAB Function6/30(u30)  "<Value_1478>"
  BUS_HD2/31 -> MATLAB Function6/31(u31)  "<Value_1488>"
  BUS_HD2/32 -> MATLAB Function6/32(u32)  "<Value_1509>"
  BUS_HD2/33 -> MATLAB Function6/33(u33)  "<Value_1522>"
  BUS_HD2/34 -> MATLAB Function6/34(u34)  "<Value_1537>"
  BUS_HD2/35 -> MATLAB Function6/35(u35)  "<Value_1550>"
  BUS_HD2/36 -> MATLAB Function6/36(u36)  "<Value_1563>"
  BUS_HD2/37 -> MATLAB Function6/37(u37)  "<Value_1576>"
  BUS_HD2/38 -> MATLAB Function6/38(u38)  "<Value_1589>"
  BUS_HD2/39 -> MATLAB Function6/39(u39)  "<Value_1602>"
  BUS_HD2/40 -> MATLAB Function6/40(u40)  "<Value_1615>"
  BUS_HD2/41 -> MATLAB Function6/41(u41)  "<Value_1628>"
  BUS_HD2/42 -> MATLAB Function6/42(u42)  "<Value_1641>"
  BUS_HD2/43 -> MATLAB Function6/43(u43)  "<Value_1654>"
  BUS_HD2/44 -> MATLAB Function6/44(u44)  "<Value_1667>"
  BUS_HD2/45 -> MATLAB Function6/45(u45)  "<Value_1680>"
  BUS_HD2/46 -> MATLAB Function6/46(u46)  "<Value_1693>"
  BUS_PROC/1 -> MATLAB Function7/1(u1)  "<Value_1204>"
  BUS_PROC/2 -> MATLAB Function7/2(u2)  "<Value_1214>"
  BUS_PROC/3 -> MATLAB Function7/3(u3)  "<Value_1224>"
  BUS_PROC/4 -> MATLAB Function7/4(u4)  "<Value_1234>"
  BUS_PROC/5 -> MATLAB Function7/5(u5)  "<Value_1244>"
  BUS_PROC/6 -> MATLAB Function7/6(u6)  "<Value_1254>"
  BUS_PROC/7 -> MATLAB Function7/7(u7)  "<Value_1264>"
  BUS_PROC/8 -> MATLAB Function7/8(u8)  "<Value_1274>"
  BUS_PROC/9 -> MATLAB Function7/9(u9)  "<Value_1284>"
  BUS_PROC/10 -> MATLAB Function7/10(u10)  "<Value_1294>"
  BUS_PROC/11 -> MATLAB Function7/11(u11)  "<Value_1310>"
  BUS_PROC/12 -> MATLAB Function7/12(u12)  "<Value_1320>"
  BUS_PROC/13 -> MATLAB Function7/13(u13)  "<Value_1330>"
  BUS_PROC/14 -> MATLAB Function7/14(u14)  "<Value_1340>"
  BUS_PROC/15 -> MATLAB Function7/15(u15)  "<Value_1350>"
  BUS_PROC/16 -> MATLAB Function7/16(u16)  "<Value_1360>"
  BUS_PROC/17 -> MATLAB Function7/17(u17)  "<Value_1370>"
  BUS_PROC/18 -> MATLAB Function7/18(u18)  "<Value_1380>"
  BUS_PROC/19 -> MATLAB Function7/19(u19)  "<Value_1390>"
  BUS_PROC/20 -> MATLAB Function7/20(u20)  "<Value_1400>"
  BUS_PROC/21 -> MATLAB Function7/21(u21)  "<Value_1410>"
  BUS_PROC/22 -> MATLAB Function7/22(u22)  "<Value_1420>"
  BUS_PROC/23 -> MATLAB Function7/23(u23)  "<Value_1430>"
  BUS_PROC/24 -> MATLAB Function7/24(u24)  "<Value_1440>"
  BUS_PROC/25 -> MATLAB Function7/25(u25)  "<Value_1461>"
  BUS_PROC/26 -> MATLAB Function7/26(u26)  "<Value_1474>"
  BUS_PROC/27 -> MATLAB Function7/27(u27)  "<Value_1489>"
  BUS_PROC/28 -> MATLAB Function7/28(u28)  "<Value_1502>"
  BUS_PROC/29 -> MATLAB Function7/29(u29)  "<Value_1515>"
  BUS_PROC/30 -> MATLAB Function7/30(u30)  "<Value_1528>"
  BUS_PROC/31 -> MATLAB Function7/31(u31)  "<Value_1541>"
  BUS_PROC/32 -> MATLAB Function7/32(u32)  "<Value_1554>"
  BUS_PROC/33 -> MATLAB Function7/33(u33)  "<Value_1567>"
  BUS_PROC/34 -> MATLAB Function7/34(u34)  "<Value_1580>"
  BUS_PROC/35 -> MATLAB Function7/35(u35)  "<Value_1593>"
  BUS_PROC/36 -> MATLAB Function7/36(u36)  "<Value_1606>"
  BUS_PROC/37 -> MATLAB Function7/37(u37)  "<Value_1619>"
  BUS_PROC/38 -> MATLAB Function7/38(u38)  "<Value_1632>"
  BUS_PROC/39 -> MATLAB Function7/39(u39)  "<Value_1645>"
  BUS_NODE/1 -> MATLAB Function1/1(u1)  "<Value_1245>"
  BUS_NODE/2 -> MATLAB Function1/2(u2)  "<Value_1255>"
  BUS_NODE/3 -> MATLAB Function1/3(u3)  "<Value_1265>"
  BUS_NODE/4 -> MATLAB Function1/4(u4)  "<Value_1275>"
  BUS_NODE/5 -> MATLAB Function1/5(u5)  "<Value_1285>"
  BUS_NODE/6 -> MATLAB Function1/6(u6)  "<Value_1295>"
  BUS_NODE/7 -> MATLAB Function1/7(u7)  "<Value_1305>"
  BUS_NODE/8 -> MATLAB Function1/8(u8)  "<Value_1315>"
  BUS_NODE/9 -> MATLAB Function1/9(u9)  "<Value_1325>"
  BUS_NODE/10 -> MATLAB Function1/10(u10)  "<Value_1335>"
  BUS_NODE/11 -> MATLAB Function1/11(u11)  "<Value_1345>"
  BUS_NODE/12 -> MATLAB Function1/12(u12)  "<Value_1355>"
  BUS_NODE/13 -> MATLAB Function1/13(u13)  "<Value_1384>"
  BUS_NODE/14 -> MATLAB Function1/14(u14)  "<Value_1397>"
  BUS_NODE/15 -> MATLAB Function1/15(u15)  "<Value_1371>"
  BUS_NODE/16 -> MATLAB Function1/16(u16)  "<Value_1413>"
  BUS_NODE/17 -> MATLAB Function1/17(u17)  "<Value_1423>"
  BUS_NODE/18 -> MATLAB Function1/18(u18)  "<Value_1433>"
  BUS_NODE/19 -> MATLAB Function1/19(u19)  "<Value_1443>"
  BUS_NODE/20 -> MATLAB Function1/20(u20)  "<Value_1453>"
  BUS_NODE/21 -> MATLAB Function1/21(u21)  "<Value_1463>"
  BUS_NODE/22 -> MATLAB Function1/22(u22)  "<Value_1599>"
  BUS_NODE/23 -> MATLAB Function1/23(u23)  "<Value_1612>"
  BUS_NODE/24 -> MATLAB Function1/24(u24)  "<Value_1625>"
  BUS_NODE/25 -> MATLAB Function1/25(u25)  "<Value_1638>"
  BUS_NODE/26 -> MATLAB Function1/26(u26)  "<Value_1651>"
  BUS_NODE/27 -> MATLAB Function1/27(u27)  "<Value_1664>"
  BUS_NODE/28 -> MATLAB Function1/28(u28)  "<Value_1677>"
  BUS_NODE/29 -> MATLAB Function1/29(u29)  "<Value_1690>"
  BUS_NODE/30 -> MATLAB Function1/30(u30)  "<Value_1703>"
  BUS_NODE/31 -> MATLAB Function1/31(u31)  "<Value_1716>"
  BUS_NODE/32 -> MATLAB Function1/32(u32)  "<Value_1729>"
  BUS_NODE/33 -> MATLAB Function1/33(u33)  "<Value_1742>"
  BUS_NODE/34 -> MATLAB Function1/34(u34)  "<Value_2551>"
  BUS_NODE/35 -> MATLAB Function1/35(u35)  "<Value_2561>"
  BUS_NODE/36 -> MATLAB Function1/36(u36)  "<Value_2571>"
  BUS_NODE/37 -> MATLAB Function1/37(u37)  "<Value_2581>"
  BUS_NODE/38 -> MATLAB Function1/38(u38)  "<Value_2591>"
  BUS_NODE/39 -> MATLAB Function1/39(u39)  "<Value_2601>"
  BUS_NODE/40 -> MATLAB Function1/40(u40)  "<Value_2611>"
  BUS_NODE/41 -> MATLAB Function1/41(u41)  "<Value_2621>"
  BUS_NODE/42 -> MATLAB Function1/42(u42)  "<Value_2631>"
  BUS_NODE/43 -> MATLAB Function1/43(u43)  "<Value_2641>"
  BUS_NODE/44 -> MATLAB Function1/44(u44)  "<Value_2651>"
  BUS_NODE/45 -> MATLAB Function1/45(u45)  "<Value_2661>"
  BUS_NODE/46 -> MATLAB Function1/46(u46)  "<Value_2677>"
  BUS_NODE/47 -> MATLAB Function1/47(u47)  "<Value_2687>"
  BUS_NODE/48 -> MATLAB Function1/48(u48)  "<Value_2697>"
  BUS_NODE/49 -> MATLAB Function1/49(u49)  "<Value_2707>"
  BUS_NODE/50 -> MATLAB Function1/50(u50)  "<Value_2717>"
  BUS_NODE/51 -> MATLAB Function1/51(u51)  "<Value_2733>"
  BUS_NODE/52 -> MATLAB Function1/52(u52)  "<Value_2743>"
  BUS_NODE/53 -> MATLAB Function1/53(u53)  "<Value_2753>"
  BUS_NODE/54 -> MATLAB Function1/54(u54)  "<Value_2763>"
  BUS_NODE/55 -> MATLAB Function1/55(u55)  "<Value_2773>"
  BUS_NODE/56 -> MATLAB Function1/56(u56)  "<Value_2783>"
  BUS_NODE/57 -> MATLAB Function1/57(u57)  "<Value_2793>"
  BUS_NODE/58 -> MATLAB Function1/58(u58)  "<Value_2803>"
  BUS_NODE/59 -> MATLAB Function1/59(u59)  "<Value_2822>"
  BUS_NODE/60 -> MATLAB Function1/60(u60)  "<Value_2835>"
  BUS_NODE/61 -> MATLAB Function1/61(u61)  "<Value_2848>"
  BUS_NODE/62 -> MATLAB Function1/62(u62)  "<Value_2861>"
  BUS_NODE/63 -> MATLAB Function1/63(u63)  "<Value_2874>"
  BUS_NODE/64 -> MATLAB Function1/64(u64)  "<Value_2887>"
  BUS_NODE/65 -> MATLAB Function1/65(u65)  "<Value_2900>"
  BUS_NODE/66 -> MATLAB Function1/66(u66)  "<Value_2913>"
